simulink model "ZT_VehCtrl_18B_CAN"  (R2018b)
settings: Solver=FixedStepAuto  StartTime=0.0  StopTime=inf  FixedStep=0.005  RelTol=1e-3
InitFcn:
  | mbd_mpc_consistency_checks(bdroot(gcs));
values from neighbouring files (symbols this model uses):
  BatoverTempTh = single(80)    [VCU_INIT.m]
  BRS_PwrValid = single(5)    [VCU_INIT.m]
  BRSEnSpdTh1 = single(10)    [VCU_INIT.m]
  BRSEnSpdTh2 = single(20)    [VCU_INIT.m]
  MCUTempAlarmTh = single (60)    [VCU_INIT.m]
  mps2kmh = single(3.6)    [VCU_INIT.m]
  MtrPwrFac = single(1/9550)    [VCU_INIT.m]
  MtrTempAlarmTh = single (50)    [VCU_INIT.m]
  Padle1Signal1_Th = [PadleSignal1_min,PadleSignal1_max]    [VCU_INIT.m]
  Padle1Signal2_Th = [PadleSignal2_min,PadleSignal2_max]    [VCU_INIT.m]
  PadleSignal1_max = 3.84    [VCU_INIT.m]
  PadleSignal1_min = 0.75    [VCU_INIT.m]
  PadleSignal2_max = 1.92    [VCU_INIT.m]
  PadleSignal2_min = 0.375    [VCU_INIT.m]
  PadleValid = 0.05    [VCU_INIT.m]
  PwrLimFactor = single(0.5)    [VCU_INIT.m]
  Ratio = single(1)    [VCU_INIT.m]
  rpm2mps = single(2*pi/60 * WhlRadius/Ratio)    [VCU_INIT.m]
  SOCLowTh = single(20)    [VCU_INIT.m]
  VehPwrBackwardMax = VehPwrMax * single(0.3)    [VCU_INIT.m]
  VehPwrMax = single(MtrPwrMax * 4)    [VCU_INIT.m]
  VehTrqBackwardMax = VehTrqMax * single(0.3)    [VCU_INIT.m]
  VehTrqMax = single(MtrTrqMax * Ratio *4)    [VCU_INIT.m]
  WhlRadius = single(1)    [VCU_INIT.m]
undefined symbols (not defined in the file or in its folder): Delay_Charge, Delay_Discharge, fifo_0_vect, fifo_1_vect, LQFP, pts1_fifo_0_vect, pts1_fifo_1_vect, pts2_fifo_0_vect, pts2_fifo_1_vect, pts3_fifo_0_vect, pts3_fifo_1_vect, pts4_fifo_0_vect, pts4_fifo_1_vect
libraries: mbd_mpc574x_ec_toolbox x157, canmsglib x74, simulink x38
(part 1 of 12)
settings Model: Creator=DELL  LastModifiedBy=22654
settings SolverCC: AutoInsertRateTranBlk=on
settings DataIOCC: ExternalInput=off  InitialState=off  SaveOutput=off  SignalLogging=off  SaveTime=off  ReturnWorkspaceOutputs=on
settings OptimizationCC: DefaultParameterBehavior=Inlined  DefaultUnderspecifiedDataType=single  EnhancedBackFolding=on  PassReuseOutputArgsAs=Individual arguments  OptimizeBlockOrder=speed  DifferentSizesBufferReuse=on  OptimizationCustomize=off
settings DebuggingCC: InheritedTsInSrcMsg=none  SingleTaskRateTransMsg=error  ParameterTunabilityLossMsg=error  UnconnectedOutputMsg=none  UnconnectedLineMsg=none  UnknownTsInhSupMsg=error  SimStateInterfaceChecksumMismatchMsg=none  UnderSpecifiedDimensionMsg=warning
settings HardwareCC: ProdBitPerPointer=32  ProdBitPerSizeT=32  ProdBitPerPtrDiffT=32  ProdLargestAtomicInteger=Long  ProdLargestAtomicFloat=Double  ProdEndianess=BigEndian  ProdWordSize=32  ProdHWDeviceType=Motorola PowerPC
settings SFSimCC: MATLABDynamicMemAlloc=off
settings RTWCC: SystemTargetFile=mbd_mpc574x.tlc  MakeCommand=mbd_mpc574x_make_rtw  TemplateMakefile=mbd_mpc574x.tmf  Description=Model Based Design Toolbox MPC57xx Code Generation Target  GenerateReport=on  IncludeHyperlinkInReport=on  LaunchReport=on  GenerateTraceInfo=on  GenerateTraceReport=on  GenerateTraceReportSl=on  GenerateTraceReportSf=on  GenerateTraceReportEml=on  RTWCompilerOptimization=on
settings CodeAppCC: ForceParamTrailComments=on  IgnoreCustomStorageClasses=off  MaxIdLength=95  OperatorAnnotations=on  SimulinkDataObjDesc=on  SFDataObjDesc=on  InsertBlockDesc=on
settings STFCustomTargetCC: TargetLangStandard=C99 (ISO)  MultiwordLength=256  CombineOutputUpdateFcns=on  ERTCustomFileBanners=on  SupportNonInlinedSFcns=off  RemoveResetFunc=on  MATLABClassNameForMDSCustomization=Simulink.SoftwareTarget.ERTCustomization  SystemTargetFile=mbd_mpc574x.tlc
settings ERTTargetCC: TargetLangStandard=C99 (ISO)  ParMdlRefBuildCompliant=off  CompOptLevelCompliant=off  ConcurrentExecutionCompliant=off  SupportContinuousTime=on  ModelStepFunctionPrototypeControlCompliant=off  CPPClassGenCompliant=off  UseToolchainInfoCompliant=off  InlinedParameterPlacement=NonHierarchical  ERTSrcFileBannerTemplate=mbd_ert_code_template.cgt  ERTHdrFileBannerTemplate=mbd_ert_code_template.cgt  ERTDataSrcFileTemplate=mbd_ert_code_template.cgt  ERTDataHdrFileTemplate=mbd_ert_code_template.cgt  ERTCustomFileTemplate=example_file_process.tlc

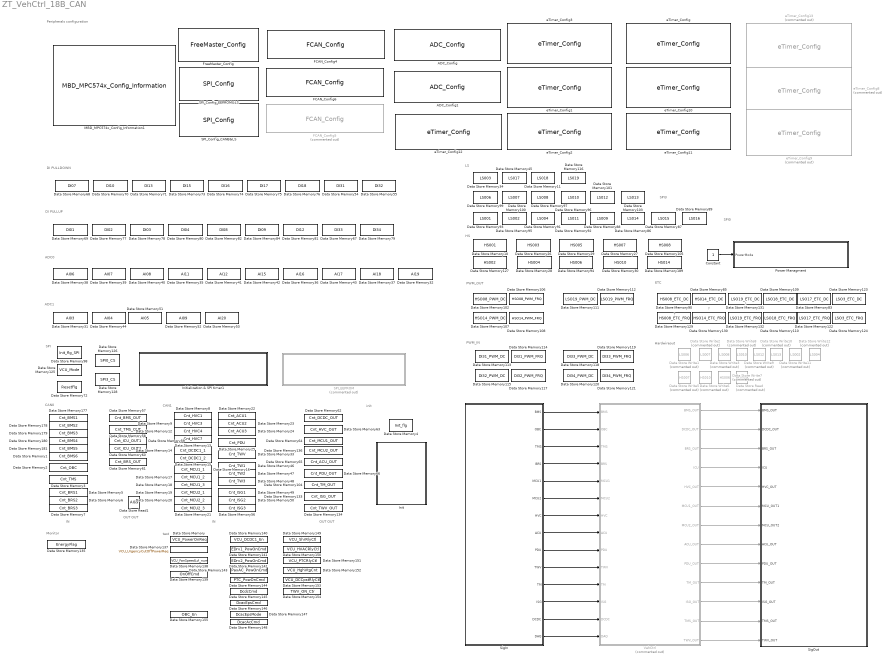
== system ZT_VehCtrl_18B_CAN ==
  note: test
  note: Monitor
  note: IN
  note: CAN1
  note: CAN0
  note: SPI0
  note: SPI3
  note: Hardwireout
  note: ?
  note: LS
  note: ETC
  note: SPI
  note: Peripherals configuration
  note: ADC1
  note: DI PULLUP
  note: PWM_OUT
  note: ADC0
  note: PWM_IN
  note: DI PULLDOWN
  note: ?
  note: ?
  note: HS
  note: init
  note: OUT
      | OUT
  note: IN
  note: OUT
      | OUT
  ADC_Config : mbd_mpc574x_ec_toolbox/Motor Control Blocks/ADC Blocks/ADC_Config  adc_instance=0  adc_mode=One-shot  adc_ctu=Disabled  adc_channels_no_n=10  adc_channel_n_0=PTC2: [ADC0_AN3 | Analog function AN3 of ADC0]  adc_channel_n_1=PTE2: [ADC0_AN5 | Analog function AN5 of ADC0]  adc_channel_n_2=PTB8: [ADC0_AN1 | Analog function AN1 of ADC0]  adc_channel_n_3=PTE7: [ADC0_AN6 | Analog function AN6 of ADC0]  adc_channel_n_4=PTB9: [ADC0_AN11 | Analog function AN11 of ADC0]  adc_channel_n_5=PTC1: [ADC0_AN2 | Analog function AN2 of ADC0]  adc_channel_n_6=PTE4: [ADC0_AN7 | Analog function AN7 of ADC0]  adc_channel_n_7=PTB7: [ADC0_AN0 | Analog function AN0 of ADC0]  adc_channel_n_8=PTE6: [ADC0_AN4 | Analog function AN4 of ADC0]  adc_channel_n_9=PTE5: [ADC0_AN8 | Analog function AN8 of ADC0]  adc_channel_n_10=not available  adc_channel_n_11=not available  adc_channel_n_12=not available  adc_channel_n_13=not available  adc_channel_n_14=not available  adc_channel_n_15=not available  adc_channel_n_16=not available  adc_channel_n_17=not available  adc_channel_n_18=not available  adc_channel_n_19=not available  adc_channel_n_20=not available  adc_channel_n_21=not available  adc_channel_n_22=not available  adc_channel_n_23=not available  adc_channel_n_24=not available  adc_channel_n_25=not available  adc_channel_n_26=not available  adc_channel_n_27=not available  adc_channel_n_28=not available  adc_channel_n_29=not available  adc_channel_n_30=not available  adc_channel_n_31=not available  adc_channel_n_32=not available  adc_channel_n_33=not available  adc_channel_n_34=not available  adc_channel_n_35=not available  adc_channel_n_36=not available  adc_channel_n_37=not available  adc_channel_n_38=not available  adc_channel_n_39=not available  adc_channel_n_40=not available  adc_channel_n_41=not available  adc_channel_n_42=not available  adc_channel_n_43=not available  adc_channel_n_44=not available  adc_channel_n_45=not available  adc_channel_n_46=not available  adc_channel_n_47=not available  show_adv_opts=on  adc_prec=100  adc_presample_0=High voltage ground for ADC  adc_int=100  adc_presample_1=High voltage ground for ADC  adc_ext=100  adc_presample_2=High voltage ground for ADC  adc_clk=Equal to bus clock  adc_ack=off  adc_ext_trigger=External Trigger Disabled  adc_skip_sampling=off  adc_calibration=on  adc_wls=Right  adc_owr=off  adc_inj_trigger=Injected Trigger Disabled  adc_mux_delay=0  adc_decode_delay=0  adc_thr_reg_no=0  adc_upper_value_0=0  adc_lower_value_0=0  adc_upper_value_1=0  adc_lower_value_1=0  adc_upper_value_2=0  adc_lower_value_2=0  adc_upper_value_3=0  adc_lower_value_3=0  adc_upper_value_4=0  adc_lower_value_4=0  adc_upper_value_5=0  adc_lower_value_5=0  adc_upper_value_6=0  adc_lower_value_6=0  adc_upper_value_7=0  adc_lower_value_7=0  adc_upper_value_8=0  adc_lower_value_8=0  adc_upper_value_9=0  adc_lower_value_9=0  adc_upper_value_10=0  adc_lower_value_10=0  adc_upper_value_11=0  adc_lower_value_11=0  adc_upper_value_12=0  adc_lower_value_12=0  adc_upper_value_13=0  adc_lower_value_13=0  adc_upper_value_14=0  adc_lower_value_14=0  adc_upper_value_15=0  adc_lower_value_15=0  adc_wdt_isr_init=off  adc_en_wdt_0=off  adc_th_index_0=0  adc_en_wdt_1=off  adc_th_index_1=0  adc_en_wdt_2=off  adc_th_index_2=0  adc_en_wdt_3=off  adc_th_index_3=0  adc_en_wdt_4=off  adc_th_index_4=0  adc_en_wdt_5=off  adc_th_index_5=0  adc_en_wdt_6=off  adc_th_index_6=0  adc_en_wdt_7=off  adc_th_index_7=0  adc_en_wdt_8=off  adc_th_index_8=0  adc_en_wdt_9=off  adc_th_index_9=0  adc_en_wdt_10=off  adc_th_index_10=0  adc_en_wdt_11=off  adc_th_index_11=0  adc_en_wdt_12=off  adc_th_index_12=0  adc_en_wdt_13=off  adc_th_index_13=0  adc_en_wdt_14=off  adc_th_index_14=0  adc_en_wdt_15=off  adc_th_index_15=0  adc_en_wdt_16=off  adc_th_index_16=0  adc_en_wdt_17=off  adc_th_index_17=0  adc_en_wdt_18=off  adc_th_index_18=0  adc_en_wdt_19=off  adc_th_index_19=0  adc_en_wdt_20=off  adc_th_index_20=0  adc_en_wdt_21=off  adc_th_index_21=0  adc_en_wdt_22=off  adc_th_index_22=0  adc_en_wdt_23=off  adc_th_index_23=0  adc_en_wdt_24=off  adc_th_index_24=0  adc_en_wdt_25=off  adc_th_index_25=0  adc_en_wdt_26=off  adc_th_index_26=0  adc_en_wdt_27=off  adc_th_index_27=0  adc_en_wdt_28=off  adc_th_index_28=0  adc_en_wdt_29=off  adc_th_index_29=0  adc_en_wdt_30=off  adc_th_index_30=0  adc_en_wdt_31=off  adc_th_index_31=0  adc_en_wdt_32=off  adc_th_index_32=0  adc_en_wdt_33=off  adc_th_index_33=0  adc_en_wdt_34=off  adc_th_index_34=0  adc_en_wdt_35=off  adc_th_index_35=0  adc_en_wdt_36=off  adc_th_index_36=0  adc_en_wdt_37=off  adc_th_index_37=0  adc_en_wdt_38=off  adc_th_index_38=0  adc_en_wdt_39=off  adc_th_index_39=0  adc_en_wdt_40=off  adc_th_index_40=0  adc_en_wdt_41=off  adc_th_index_41=0  adc_en_wdt_42=off  adc_th_index_42=0  adc_en_wdt_43=off  adc_th_index_43=0  adc_en_wdt_44=off  adc_th_index_44=0  adc_en_wdt_45=off  adc_th_index_45=0  adc_en_wdt_46=off  adc_th_index_46=0  adc_en_wdt_47=off  adc_th_index_47=0
  ADC_Config1 : mbd_mpc574x_ec_toolbox/Motor Control Blocks/ADC Blocks/ADC_Config  adc_instance=1  adc_mode=One-shot  adc_ctu=Disabled  adc_channels_no_n=5  adc_channel_n_0=PTC0: [ADC1_AN3 | Analog function AN3 of ADC1]  adc_channel_n_1=PTE11: [ADC1_AN4 | Analog function AN4 of ADC1]  adc_channel_n_2=PTB15: [ADC1_AN2 | Analog function AN2 of ADC1]  adc_channel_n_3=PTE0: [ADC1_AN5 | Analog function AN5 of ADC1]  adc_channel_n_4=PTB14: [ADC1_AN1 | Analog function AN1 of ADC1]  adc_channel_n_5=not available  adc_channel_n_6=not available  adc_channel_n_7=not available  adc_channel_n_8=not available  adc_channel_n_9=not available  adc_channel_n_10=not available  adc_channel_n_11=not available  adc_channel_n_12=not available  adc_channel_n_13=not available  adc_channel_n_14=not available  adc_channel_n_15=not available  adc_channel_n_16=not available  adc_channel_n_17=not available  adc_channel_n_18=not available  adc_channel_n_19=not available  adc_channel_n_20=not available  adc_channel_n_21=not available  adc_channel_n_22=not available  adc_channel_n_23=not available  adc_channel_n_24=not available  adc_channel_n_25=not available  adc_channel_n_26=not available  adc_channel_n_27=not available  adc_channel_n_28=not available  adc_channel_n_29=not available  adc_channel_n_30=not available  adc_channel_n_31=not available  adc_channel_n_32=not available  adc_channel_n_33=not available  adc_channel_n_34=not available  adc_channel_n_35=not available  adc_channel_n_36=not available  adc_channel_n_37=not available  adc_channel_n_38=not available  adc_channel_n_39=not available  adc_channel_n_40=not available  adc_channel_n_41=not available  adc_channel_n_42=not available  adc_channel_n_43=not available  adc_channel_n_44=not available  adc_channel_n_45=not available  adc_channel_n_46=not available  adc_channel_n_47=not available  show_adv_opts=on  adc_prec=100  adc_presample_0=High voltage ground for ADC  adc_int=100  adc_presample_1=High voltage ground for ADC  adc_ext=100  adc_presample_2=High voltage ground for ADC  adc_clk=Equal to bus clock  adc_ack=off  adc_ext_trigger=External Trigger Disabled  adc_skip_sampling=off  adc_calibration=on  adc_wls=Right  adc_owr=off  adc_inj_trigger=Injected Trigger Disabled  adc_mux_delay=0  adc_decode_delay=0  adc_thr_reg_no=0  adc_upper_value_0=0  adc_lower_value_0=0  adc_upper_value_1=0  adc_lower_value_1=0  adc_upper_value_2=0  adc_lower_value_2=0  adc_upper_value_3=0  adc_lower_value_3=0  adc_upper_value_4=0  adc_lower_value_4=0  adc_upper_value_5=0  adc_lower_value_5=0  adc_upper_value_6=0  adc_lower_value_6=0  adc_upper_value_7=0  adc_lower_value_7=0  adc_upper_value_8=0  adc_lower_value_8=0  adc_upper_value_9=0  adc_lower_value_9=0  adc_upper_value_10=0  adc_lower_value_10=0  adc_upper_value_11=0  adc_lower_value_11=0  adc_upper_value_12=0  adc_lower_value_12=0  adc_upper_value_13=0  adc_lower_value_13=0  adc_upper_value_14=0  adc_lower_value_14=0  adc_upper_value_15=0  adc_lower_value_15=0  adc_wdt_isr_init=off  adc_en_wdt_0=off  adc_th_index_0=0  adc_en_wdt_1=off  adc_th_index_1=0  adc_en_wdt_2=off  adc_th_index_2=0  adc_en_wdt_3=off  adc_th_index_3=0  adc_en_wdt_4=off  adc_th_index_4=0  adc_en_wdt_5=off  adc_th_index_5=0  adc_en_wdt_6=off  adc_th_index_6=0  adc_en_wdt_7=off  adc_th_index_7=0  adc_en_wdt_8=off  adc_th_index_8=0  adc_en_wdt_9=off  adc_th_index_9=0  adc_en_wdt_10=off  adc_th_index_10=0  adc_en_wdt_11=off  adc_th_index_11=0  adc_en_wdt_12=off  adc_th_index_12=0  adc_en_wdt_13=off  adc_th_index_13=0  adc_en_wdt_14=off  adc_th_index_14=0  adc_en_wdt_15=off  adc_th_index_15=0  adc_en_wdt_16=off  adc_th_index_16=0  adc_en_wdt_17=off  adc_th_index_17=0  adc_en_wdt_18=off  adc_th_index_18=0  adc_en_wdt_19=off  adc_th_index_19=0  adc_en_wdt_20=off  adc_th_index_20=0  adc_en_wdt_21=off  adc_th_index_21=0  adc_en_wdt_22=off  adc_th_index_22=0  adc_en_wdt_23=off  adc_th_index_23=0  adc_en_wdt_24=off  adc_th_index_24=0  adc_en_wdt_25=off  adc_th_index_25=0  adc_en_wdt_26=off  adc_th_index_26=0  adc_en_wdt_27=off  adc_th_index_27=0  adc_en_wdt_28=off  adc_th_index_28=0  adc_en_wdt_29=off  adc_th_index_29=0  adc_en_wdt_30=off  adc_th_index_30=0  adc_en_wdt_31=off  adc_th_index_31=0  adc_en_wdt_32=off  adc_th_index_32=0  adc_en_wdt_33=off  adc_th_index_33=0  adc_en_wdt_34=off  adc_th_index_34=0  adc_en_wdt_35=off  adc_th_index_35=0  adc_en_wdt_36=off  adc_th_index_36=0  adc_en_wdt_37=off  adc_th_index_37=0  adc_en_wdt_38=off  adc_th_index_38=0  adc_en_wdt_39=off  adc_th_index_39=0  adc_en_wdt_40=off  adc_th_index_40=0  adc_en_wdt_41=off  adc_th_index_41=0  adc_en_wdt_42=off  adc_th_index_42=0  adc_en_wdt_43=off  adc_th_index_43=0  adc_en_wdt_44=off  adc_th_index_44=0  adc_en_wdt_45=off  adc_th_index_45=0  adc_en_wdt_46=off  adc_th_index_46=0  adc_en_wdt_47=off  adc_th_index_47=0
  Constant : Constant
  Data Store Memory : DataStoreMemory  DataStoreName=VCU_PowerOnReq  ReadBeforeWriteMsg=warning  WriteAfterWriteMsg=warning  WriteAfterReadMsg=warning  ShowAdditionalParam=off  OutDataTypeStr=boolean
      settings: RTWStateStorageClass=ExportedGlobal
  Data Store Memory1 : DataStoreMemory  DataStoreName=Cnt_BMS6  ReadBeforeWriteMsg=warning  WriteAfterWriteMsg=warning  WriteAfterReadMsg=warning  ShowAdditionalParam=off  OutDataTypeStr=uint8
      settings: RTWStateStorageClass=ExportedGlobal
  Data Store Memory10 : DataStoreMemory  DataStoreName=HS001  ReadBeforeWriteMsg=warning  WriteAfterWriteMsg=warning  WriteAfterReadMsg=warning  ShowAdditionalParam=off  OutDataTypeStr=boolean
  Data Store Memory100 : DataStoreMemory  DataStoreName=LS007  ReadBeforeWriteMsg=warning  WriteAfterWriteMsg=warning  WriteAfterReadMsg=warning  ShowAdditionalParam=off  OutDataTypeStr=boolean
      settings: RTWStateStorageClass=ExportedGlobal
  Data Store Memory101 : DataStoreMemory  DataStoreName=LS012  ReadBeforeWriteMsg=warning  WriteAfterWriteMsg=warning  WriteAfterReadMsg=warning  ShowAdditionalParam=off  OutDataTypeStr=boolean
      settings: RTWStateStorageClass=ExportedGlobal
  Data Store Memory102 : DataStoreMemory  DataStoreName=HSO08_PWM_DC  ReadBeforeWriteMsg=warning  WriteAfterWriteMsg=warning  WriteAfterReadMsg=warning  ShowAdditionalParam=off  OutMin=0  OutMax=1  OutDataTypeStr=single
  Data Store Memory103 : DataStoreMemory  DataStoreName=LS013  ReadBeforeWriteMsg=warning  WriteAfterWriteMsg=warning  WriteAfterReadMsg=warning  ShowAdditionalParam=off  OutDataTypeStr=boolean
      settings: RTWStateStorageClass=ExportedGlobal
  Data Store Memory104 : DataStoreMemory  DataStoreName=Cnt_TM_OUT  ReadBeforeWriteMsg=warning  WriteAfterWriteMsg=warning  WriteAfterReadMsg=warning  ShowAdditionalParam=off  OutDataTypeStr=uint8
      settings: RTWStateStorageClass=ExportedGlobal
  Data Store Memory105 : DataStoreMemory  DataStoreName=HS008  ReadBeforeWriteMsg=warning  WriteAfterWriteMsg=warning  WriteAfterReadMsg=warning  ShowAdditionalParam=off  OutDataTypeStr=boolean
  Data Store Memory106 : DataStoreMemory  DataStoreName=HSO08_PWM_FRQ  ReadBeforeWriteMsg=warning  WriteAfterWriteMsg=warning  WriteAfterReadMsg=warning  InitialValue=200  ShowAdditionalParam=off  OutMin=20  OutMax=20000  OutDataTypeStr=single
  Data Store Memory107 : DataStoreMemory  DataStoreName=HSO14_PWM_DC  ReadBeforeWriteMsg=warning  WriteAfterWriteMsg=warning  WriteAfterReadMsg=warning  ShowAdditionalParam=off  OutMin=0  OutMax=1  OutDataTypeStr=single
  Data Store Memory108 : DataStoreMemory  DataStoreName=HSO14_PWM_FRQ  ReadBeforeWriteMsg=warning  WriteAfterWriteMsg=warning  WriteAfterReadMsg=warning  InitialValue=200  ShowAdditionalParam=off  OutMin=20  OutMax=20000  OutDataTypeStr=single
  Data Store Memory109 : DataStoreMemory  DataStoreName=LSO18_ETC_DC  ReadBeforeWriteMsg=warning  WriteAfterWriteMsg=warning  WriteAfterReadMsg=warning  ShowAdditionalParam=off  OutMin=0  OutMax=1  OutDataTypeStr=single
  Data Store Memory11 : DataStoreMemory  DataStoreName=LS018  ReadBeforeWriteMsg=warning  WriteAfterWriteMsg=warning  WriteAfterReadMsg=warning  ShowAdditionalParam=off  OutDataTypeStr=boolean
      settings: RTWStateStorageClass=ExportedGlobal
  Data Store Memory110 : DataStoreMemory  DataStoreName=LSO18_ETC_FRQ  ReadBeforeWriteMsg=warning  WriteAfterWriteMsg=warning  WriteAfterReadMsg=warning  InitialValue=200  ShowAdditionalParam=off  OutMin=20  OutMax=20000  OutDataTypeStr=single
  Data Store Memory111 : DataStoreMemory  DataStoreName=LSO19_PWM_DC  ReadBeforeWriteMsg=warning  WriteAfterWriteMsg=warning  WriteAfterReadMsg=warning  ShowAdditionalParam=off  OutMin=0  OutMax=1  OutDataTypeStr=single
  Data Store Memory112 : DataStoreMemory  DataStoreName=LSO19_PWM_FRQ  ReadBeforeWriteMsg=warning  WriteAfterWriteMsg=warning  WriteAfterReadMsg=warning  InitialValue=200  ShowAdditionalParam=off  OutMin=20  OutMax=20000  OutDataTypeStr=single
  Data Store Memory113 : DataStoreMemory  DataStoreName=DI31_PWM_DC  ReadBeforeWriteMsg=warning  WriteAfterWriteMsg=warning  WriteAfterReadMsg=warning  InitialValue=0.5  ShowAdditionalParam=off  OutDataTypeStr=single
  Data Store Memory114 : DataStoreMemory  DataStoreName=DI31_PWM_FRQ  ReadBeforeWriteMsg=warning  WriteAfterWriteMsg=warning  WriteAfterReadMsg=warning  InitialValue=200  ShowAdditionalParam=off  OutDataTypeStr=single
  Data Store Memory115 : DataStoreMemory  DataStoreName=DI32_PWM_DC  ReadBeforeWriteMsg=warning  WriteAfterWriteMsg=warning  WriteAfterReadMsg=warning  InitialValue=0.5  ShowAdditionalParam=off  OutDataTypeStr=single
  Data Store Memory116 : DataStoreMemory  DataStoreName=LS019  ReadBeforeWriteMsg=warning  WriteAfterWriteMsg=warning  WriteAfterReadMsg=warning  ShowAdditionalParam=off  OutDataTypeStr=boolean
      settings: RTWStateStorageClass=ExportedGlobal
  Data Store Memory117 : DataStoreMemory  DataStoreName=DI32_PWM_FRQ  ReadBeforeWriteMsg=warning  WriteAfterWriteMsg=warning  WriteAfterReadMsg=warning  InitialValue=200  ShowAdditionalParam=off  OutDataTypeStr=single
  Data Store Memory118 : DataStoreMemory  DataStoreName=DI33_PWM_DC  ReadBeforeWriteMsg=warning  WriteAfterWriteMsg=warning  WriteAfterReadMsg=warning  InitialValue=0.5  ShowAdditionalParam=off  OutDataTypeStr=single
  Data Store Memory119 : DataStoreMemory  DataStoreName=DI33_PWM_FRQ  ReadBeforeWriteMsg=warning  WriteAfterWriteMsg=warning  WriteAfterReadMsg=warning  InitialValue=200  ShowAdditionalParam=off  OutDataTypeStr=single
  Data Store Memory12 : DataStoreMemory  DataStoreName=Cnt_HVC4  ReadBeforeWriteMsg=warning  WriteAfterWriteMsg=warning  WriteAfterReadMsg=warning  ShowAdditionalParam=off  OutDataTypeStr=uint8
      settings: RTWStateStorageClass=ExportedGlobal
  Data Store Memory120 : DataStoreMemory  DataStoreName=DI34_PWM_DC  ReadBeforeWriteMsg=warning  WriteAfterWriteMsg=warning  WriteAfterReadMsg=warning  InitialValue=0.5  ShowAdditionalParam=off  OutDataTypeStr=single
  Data Store Memory121 : DataStoreMemory  DataStoreName=DI34_PWM_FRQ  ReadBeforeWriteMsg=warning  WriteAfterWriteMsg=warning  WriteAfterReadMsg=warning  InitialValue=200  ShowAdditionalParam=off  OutDataTypeStr=single
  Data Store Memory122 : DataStoreMemory  DataStoreName=LSO17_ETC_FRQ  ReadBeforeWriteMsg=warning  WriteAfterWriteMsg=warning  WriteAfterReadMsg=warning  InitialValue=200  ShowAdditionalParam=off  OutMin=20  OutMax=20000  OutDataTypeStr=single
  Data Store Memory123 : DataStoreMemory  DataStoreName=LSO3_ETC_DC  ReadBeforeWriteMsg=warning  WriteAfterWriteMsg=warning  WriteAfterReadMsg=warning  ShowAdditionalParam=off  OutMin=0  OutMax=1  OutDataTypeStr=single
  Data Store Memory124 : DataStoreMemory  DataStoreName=LSO3_ETC_FRQ  ReadBeforeWriteMsg=warning  WriteAfterWriteMsg=warning  WriteAfterReadMsg=warning  InitialValue=200  ShowAdditionalParam=off  OutMin=20  OutMax=20000  OutDataTypeStr=single
  Data Store Memory125 : DataStoreMemory  DataStoreName=VCU_Mode  ReadBeforeWriteMsg=warning  WriteAfterWriteMsg=warning  WriteAfterReadMsg=warning  ShowAdditionalParam=off  OutDataTypeStr=uint8
      settings: RTWStateStorageClass=ExportedGlobal
  Data Store Memory126 : DataStoreMemory  DataStoreName=SPI0_CS  ReadBeforeWriteMsg=warning  WriteAfterWriteMsg=warning  WriteAfterReadMsg=warning  ShowAdditionalParam=off  OutDataTypeStr=boolean
  Data Store Memory127 : DataStoreMemory  DataStoreName=HS002  ReadBeforeWriteMsg=warning  WriteAfterWriteMsg=warning  WriteAfterReadMsg=warning  ShowAdditionalParam=off  OutDataTypeStr=boolean
  Data Store Memory128 : DataStoreMemory  DataStoreName=SPI3_CS  ReadBeforeWriteMsg=warning  WriteAfterWriteMsg=warning  WriteAfterReadMsg=warning  ShowAdditionalParam=off  OutDataTypeStr=boolean
  Data Store Memory129 : DataStoreMemory  DataStoreName=HS008_ETC_FRQ  ReadBeforeWriteMsg=warning  WriteAfterWriteMsg=warning  WriteAfterReadMsg=warning  InitialValue=200  ShowAdditionalParam=off  OutMin=20  OutMax=20000  OutDataTypeStr=single
  Data Store Memory13 : DataStoreMemory  DataStoreName=Cnt_HVC7  ReadBeforeWriteMsg=warning  WriteAfterWriteMsg=warning  WriteAfterReadMsg=warning  ShowAdditionalParam=off  OutDataTypeStr=uint8
      settings: RTWStateStorageClass=ExportedGlobal
  Data Store Memory130 : DataStoreMemory  DataStoreName=HSO14_ETC_FRQ  ReadBeforeWriteMsg=warning  WriteAfterWriteMsg=warning  WriteAfterReadMsg=warning  InitialValue=200  ShowAdditionalParam=off  OutMin=20  OutMax=20000  OutDataTypeStr=single
  Data Store Memory131 : DataStoreMemory  DataStoreName=LSO19_ETC_DC  ReadBeforeWriteMsg=warning  WriteAfterWriteMsg=warning  WriteAfterReadMsg=warning  ShowAdditionalParam=off  OutMin=0  OutMax=1  OutDataTypeStr=single
  Data Store Memory132 : DataStoreMemory  DataStoreName=LSO19_ETC_FRQ  ReadBeforeWriteMsg=warning  WriteAfterWriteMsg=warning  WriteAfterReadMsg=warning  InitialValue=200  ShowAdditionalParam=off  OutMin=20  OutMax=20000  OutDataTypeStr=single
  Data Store Memory133 : DataStoreMemory  DataStoreName=Cnt_ISG_OUT  ReadBeforeWriteMsg=warning  WriteAfterWriteMsg=warning  WriteAfterReadMsg=warning  ShowAdditionalParam=off  OutDataTypeStr=uint8
      settings: RTWStateStorageClass=ExportedGlobal
  Data Store Memory134 : DataStoreMemory  DataStoreName=Cnt_TWV_OUT  ReadBeforeWriteMsg=warning  WriteAfterWriteMsg=warning  WriteAfterReadMsg=warning  ShowAdditionalParam=off  OutDataTypeStr=uint8
      settings: RTWStateStorageClass=ExportedGlobal
  Data Store Memory135 : DataStoreMemory  DataStoreName=EnergyFlag  ReadBeforeWriteMsg=warning  WriteAfterWriteMsg=warning  WriteAfterReadMsg=warning  ShowAdditionalParam=off  OutDataTypeStr=uint8
      settings: RTWStateStorageClass=ExportedGlobal
  Data Store Memory136 : DataStoreMemory  DataStoreName=Cnt_MCU2_OUT  ReadBeforeWriteMsg=warning  WriteAfterWriteMsg=warning  WriteAfterReadMsg=warning  ShowAdditionalParam=off  OutDataTypeStr=uint8
      settings: RTWStateStorageClass=ExportedGlobal
  Data Store Memory137 : DataStoreMemory  DataStoreName=VCU_UrgencyCutOffPowerReq  ReadBeforeWriteMsg=warning  WriteAfterWriteMsg=warning  WriteAfterReadMsg=warning  ShowAdditionalParam=off  OutDataTypeStr=boolean
      settings: RTWStateStorageClass=ExportedGlobal
  Data Store Memory138 : DataStoreMemory  DataStoreName=VCU_FanSpeedLvl_num  ReadBeforeWriteMsg=warning  WriteAfterWriteMsg=warning  WriteAfterReadMsg=warning  ShowAdditionalParam=off  OutDataTypeStr=single
      settings: RTWStateStorageClass=ExportedGlobal
  Data Store Memory139 : DataStoreMemory  DataStoreName=OnOffCmd  ReadBeforeWriteMsg=warning  WriteAfterWriteMsg=warning  WriteAfterReadMsg=warning  ShowAdditionalParam=off  OutDataTypeStr=boolean
      settings: RTWStateStorageClass=ExportedGlobal
  Data Store Memory14 : DataStoreMemory  DataStoreName=Cnt_DCDC1_1  ReadBeforeWriteMsg=warning  WriteAfterWriteMsg=warning  WriteAfterReadMsg=warning  ShowAdditionalParam=off  OutDataTypeStr=uint8
      settings: RTWStateStorageClass=ExportedGlobal
  Data Store Memory140 : DataStoreMemory  DataStoreName=VCU_DCDC1_En  ReadBeforeWriteMsg=warning  WriteAfterWriteMsg=warning  WriteAfterReadMsg=warning  ShowAdditionalParam=off  OutDataTypeStr=single
      settings: RTWStateStorageClass=ExportedGlobal
  Data Store Memory141 : DataStoreMemory  DataStoreName=EDrv1_PowOnCmd  ReadBeforeWriteMsg=warning  WriteAfterWriteMsg=warning  WriteAfterReadMsg=warning  ShowAdditionalParam=off  OutDataTypeStr=boolean
      settings: RTWStateStorageClass=ExportedGlobal
  Data Store Memory142 : DataStoreMemory  DataStoreName=EDrv2_PowOnCmd  ReadBeforeWriteMsg=warning  WriteAfterWriteMsg=warning  WriteAfterReadMsg=warning  ShowAdditionalParam=off  OutDataTypeStr=boolean
      settings: RTWStateStorageClass=ExportedGlobal
  Data Store Memory143 : DataStoreMemory  DataStoreName=PaxAC_PowOnCmd  ReadBeforeWriteMsg=warning  WriteAfterWriteMsg=warning  WriteAfterReadMsg=warning  ShowAdditionalParam=off  OutDataTypeStr=boolean
      settings: RTWStateStorageClass=ExportedGlobal
  Data Store Memory144 : DataStoreMemory  DataStoreName=PTC_PowOnCmd  ReadBeforeWriteMsg=warning  WriteAfterWriteMsg=warning  WriteAfterReadMsg=warning  ShowAdditionalParam=off  OutDataTypeStr=boolean
      settings: RTWStateStorageClass=ExportedGlobal
  Data Store Memory145 : DataStoreMemory  DataStoreName=DcdcCmd  ReadBeforeWriteMsg=warning  WriteAfterWriteMsg=warning  WriteAfterReadMsg=warning  ShowAdditionalParam=off  OutDataTypeStr=single
      settings: RTWStateStorageClass=ExportedGlobal
  Data Store Memory146 : DataStoreMemory  DataStoreName=DcacEpsCmd  ReadBeforeWriteMsg=warning  WriteAfterWriteMsg=warning  WriteAfterReadMsg=warning  ShowAdditionalParam=off  OutDataTypeStr=single
      settings: RTWStateStorageClass=ExportedGlobal
  Data Store Memory147 : DataStoreMemory  DataStoreName=DcacEpsMode  ReadBeforeWriteMsg=warning  WriteAfterWriteMsg=warning  WriteAfterReadMsg=warning  ShowAdditionalParam=off  OutDataTypeStr=single
      settings: RTWStateStorageClass=ExportedGlobal
  Data Store Memory148 : DataStoreMemory  DataStoreName=DcacAcCmd  ReadBeforeWriteMsg=warning  WriteAfterWriteMsg=warning  WriteAfterReadMsg=warning  ShowAdditionalParam=off  OutDataTypeStr=single
      settings: RTWStateStorageClass=ExportedGlobal
  Data Store Memory149 : DataStoreMemory  DataStoreName=VCU_ShrRlyCtl  ReadBeforeWriteMsg=warning  WriteAfterWriteMsg=warning  WriteAfterReadMsg=warning  ShowAdditionalParam=off  OutDataTypeStr=single
      settings: RTWStateStorageClass=ExportedGlobal
  Data Store Memory15 : DataStoreMemory  DataStoreName=Cnt_DCDC1_2  ReadBeforeWriteMsg=warning  WriteAfterWriteMsg=warning  WriteAfterReadMsg=warning  ShowAdditionalParam=off  OutDataTypeStr=uint8
      settings: RTWStateStorageClass=ExportedGlobal
  Data Store Memory150 : DataStoreMemory  DataStoreName=VCU_HVACRlyCtl  ReadBeforeWriteMsg=warning  WriteAfterWriteMsg=warning  WriteAfterReadMsg=warning  ShowAdditionalParam=off  OutDataTypeStr=single
      settings: RTWStateStorageClass=ExportedGlobal
  Data Store Memory151 : DataStoreMemory  DataStoreName=VCU_PTCRlyCtl  ReadBeforeWriteMsg=warning  WriteAfterWriteMsg=warning  WriteAfterReadMsg=warning  ShowAdditionalParam=off  OutDataTypeStr=single
      settings: RTWStateStorageClass=ExportedGlobal
  Data Store Memory152 : DataStoreMemory  DataStoreName=VCU_HghVtgCnt  ReadBeforeWriteMsg=warning  WriteAfterWriteMsg=warning  WriteAfterReadMsg=warning  ShowAdditionalParam=off  OutDataTypeStr=single
      settings: RTWStateStorageClass=ExportedGlobal
  Data Store Memory153 : DataStoreMemory  DataStoreName=VCU_DCCpstRlyCtl  ReadBeforeWriteMsg=warning  WriteAfterWriteMsg=warning  WriteAfterReadMsg=warning  ShowAdditionalParam=off  OutDataTypeStr=single
      settings: RTWStateStorageClass=ExportedGlobal
  Data Store Memory154 : DataStoreMemory  DataStoreName=TWV_ON_Ctr  ReadBeforeWriteMsg=warning  WriteAfterWriteMsg=warning  WriteAfterReadMsg=warning  ShowAdditionalParam=off  OutDataTypeStr=single
      settings: RTWStateStorageClass=ExportedGlobal
  Data Store Memory155 : DataStoreMemory  DataStoreName=OBC_En  ReadBeforeWriteMsg=warning  WriteAfterWriteMsg=warning  WriteAfterReadMsg=warning  ShowAdditionalParam=off  OutDataTypeStr=boolean
      settings: RTWStateStorageClass=ExportedGlobal
  Data Store Memory16 : DataStoreMemory  DataStoreName=Cnt_MCU1_1  ReadBeforeWriteMsg=warning  WriteAfterWriteMsg=warning  WriteAfterReadMsg=warning  ShowAdditionalParam=off  OutDataTypeStr=uint8
      settings: RTWStateStorageClass=ExportedGlobal
  Data Store Memory17 : DataStoreMemory  DataStoreName=Cnt_MCU1_2  ReadBeforeWriteMsg=warning  WriteAfterWriteMsg=warning  WriteAfterReadMsg=warning  ShowAdditionalParam=off  OutDataTypeStr=uint8
      settings: RTWStateStorageClass=ExportedGlobal
  Data Store Memory177 : DataStoreMemory  DataStoreName=Cnt_BMS1  ReadBeforeWriteMsg=warning  WriteAfterWriteMsg=warning  WriteAfterReadMsg=warning  ShowAdditionalParam=off  OutDataTypeStr=uint8
      settings: RTWStateStorageClass=ExportedGlobal
  Data Store Memory178 : DataStoreMemory  DataStoreName=Cnt_BMS2  ReadBeforeWriteMsg=warning  WriteAfterWriteMsg=warning  WriteAfterReadMsg=warning  ShowAdditionalParam=off  OutDataTypeStr=uint8
      settings: RTWStateStorageClass=ExportedGlobal
  Data Store Memory179 : DataStoreMemory  DataStoreName=Cnt_BMS3  ReadBeforeWriteMsg=warning  WriteAfterWriteMsg=warning  WriteAfterReadMsg=warning  ShowAdditionalParam=off  OutDataTypeStr=uint8
      settings: RTWStateStorageClass=ExportedGlobal
  Data Store Memory18 : DataStoreMemory  DataStoreName=Cnt_MCU1_3  ReadBeforeWriteMsg=warning  WriteAfterWriteMsg=warning  WriteAfterReadMsg=warning  ShowAdditionalParam=off  OutDataTypeStr=uint8
      settings: RTWStateStorageClass=ExportedGlobal
  Data Store Memory180 : DataStoreMemory  DataStoreName=Cnt_BMS4  ReadBeforeWriteMsg=warning  WriteAfterWriteMsg=warning  WriteAfterReadMsg=warning  ShowAdditionalParam=off  OutDataTypeStr=uint8
      settings: RTWStateStorageClass=ExportedGlobal
  Data Store Memory181 : DataStoreMemory  DataStoreName=Cnt_BMS5  ReadBeforeWriteMsg=warning  WriteAfterWriteMsg=warning  WriteAfterReadMsg=warning  ShowAdditionalParam=off  OutDataTypeStr=uint8
      settings: RTWStateStorageClass=ExportedGlobal
  Data Store Memory189 : DataStoreMemory  DataStoreName=HS014  ReadBeforeWriteMsg=warning  WriteAfterWriteMsg=warning  WriteAfterReadMsg=warning  ShowAdditionalParam=off  OutDataTypeStr=boolean
  Data Store Memory19 : DataStoreMemory  DataStoreName=Cnt_MCU2_1  ReadBeforeWriteMsg=warning  WriteAfterWriteMsg=warning  WriteAfterReadMsg=warning  ShowAdditionalParam=off  OutDataTypeStr=uint8
      settings: RTWStateStorageClass=ExportedGlobal
  Data Store Memory2 : DataStoreMemory  DataStoreName=Cnt_OBC  ReadBeforeWriteMsg=warning  WriteAfterWriteMsg=warning  WriteAfterReadMsg=warning  ShowAdditionalParam=off  OutDataTypeStr=uint8
      settings: RTWStateStorageClass=ExportedGlobal
  Data Store Memory20 : DataStoreMemory  DataStoreName=Cnt_MCU2_2  ReadBeforeWriteMsg=warning  WriteAfterWriteMsg=warning  WriteAfterReadMsg=warning  ShowAdditionalParam=off  OutDataTypeStr=uint8
      settings: RTWStateStorageClass=ExportedGlobal
  Data Store Memory21 : DataStoreMemory  DataStoreName=Cnt_MCU2_3  ReadBeforeWriteMsg=warning  WriteAfterWriteMsg=warning  WriteAfterReadMsg=warning  ShowAdditionalParam=off  OutDataTypeStr=uint8
      settings: RTWStateStorageClass=ExportedGlobal
  Data Store Memory22 : DataStoreMemory  DataStoreName=Cnt_ACU1  ReadBeforeWriteMsg=warning  WriteAfterWriteMsg=warning  WriteAfterReadMsg=warning  ShowAdditionalParam=off  OutDataTypeStr=uint8
      settings: RTWStateStorageClass=ExportedGlobal
  Data Store Memory23 : DataStoreMemory  DataStoreName=Cnt_ACU2  ReadBeforeWriteMsg=warning  WriteAfterWriteMsg=warning  WriteAfterReadMsg=warning  ShowAdditionalParam=off  OutDataTypeStr=uint8
      settings: RTWStateStorageClass=ExportedGlobal
  Data Store Memory24 : DataStoreMemory  DataStoreName=Cnt_ACU3  ReadBeforeWriteMsg=warning  WriteAfterWriteMsg=warning  WriteAfterReadMsg=warning  ShowAdditionalParam=off  OutDataTypeStr=uint8
      settings: RTWStateStorageClass=ExportedGlobal
  Data Store Memory25 : DataStoreMemory  DataStoreName=Cnt_PDU  ReadBeforeWriteMsg=warning  WriteAfterWriteMsg=warning  WriteAfterReadMsg=warning  ShowAdditionalParam=off  OutDataTypeStr=uint8
      settings: RTWStateStorageClass=ExportedGlobal
  Data Store Memory26 : DataStoreMemory  DataStoreName=HS003  ReadBeforeWriteMsg=warning  WriteAfterWriteMsg=warning  WriteAfterReadMsg=warning  ShowAdditionalParam=off  OutDataTypeStr=boolean
  Data Store Memory27 : DataStoreMemory  DataStoreName=HS007  ReadBeforeWriteMsg=warning  WriteAfterWriteMsg=warning  WriteAfterReadMsg=warning  ShowAdditionalParam=off  OutDataTypeStr=boolean
  Data Store Memory28 : DataStoreMemory  DataStoreName=HS004  ReadBeforeWriteMsg=warning  WriteAfterWriteMsg=warning  WriteAfterReadMsg=warning  ShowAdditionalParam=off  OutDataTypeStr=boolean
  Data Store Memory29 : DataStoreMemory  DataStoreName=HS005  ReadBeforeWriteMsg=warning  WriteAfterWriteMsg=warning  WriteAfterReadMsg=warning  ShowAdditionalParam=off  OutDataTypeStr=boolean
  Data Store Memory3 : DataStoreMemory  DataStoreName=Cnt_TMS  ReadBeforeWriteMsg=warning  WriteAfterWriteMsg=warning  WriteAfterReadMsg=warning  ShowAdditionalParam=off  OutDataTypeStr=uint8
      settings: RTWStateStorageClass=ExportedGlobal
  Data Store Memory30 : DataStoreMemory  DataStoreName=HS010  ReadBeforeWriteMsg=warning  WriteAfterWriteMsg=warning  WriteAfterReadMsg=warning  ShowAdditionalParam=off  OutDataTypeStr=boolean
  Data Store Memory31 : DataStoreMemory  DataStoreName=AI03  ReadBeforeWriteMsg=warning  WriteAfterWriteMsg=warning  WriteAfterReadMsg=warning  ShowAdditionalParam=off  OutDataTypeStr=single
  Data Store Memory32 : DataStoreMemory  DataStoreName=AI19  ReadBeforeWriteMsg=warning  WriteAfterWriteMsg=warning  WriteAfterReadMsg=warning  ShowAdditionalParam=off  OutDataTypeStr=single
  Data Store Memory33 : DataStoreMemory  DataStoreName=Cnt_TWV  ReadBeforeWriteMsg=warning  WriteAfterWriteMsg=warning  WriteAfterReadMsg=warning  ShowAdditionalParam=off  OutDataTypeStr=uint8
      settings: RTWStateStorageClass=ExportedGlobal
  Data Store Memory34 : DataStoreMemory  DataStoreName=LS003  ReadBeforeWriteMsg=warning  WriteAfterWriteMsg=warning  WriteAfterReadMsg=warning  ShowAdditionalParam=off  OutDataTypeStr=boolean
      settings: RTWStateStorageClass=ExportedGlobal
  Data Store Memory35 : DataStoreMemory  DataStoreName=AI11  ReadBeforeWriteMsg=warning  WriteAfterWriteMsg=warning  WriteAfterReadMsg=warning  ShowAdditionalParam=off  OutDataTypeStr=single
  Data Store Memory36 : DataStoreMemory  DataStoreName=AI16  ReadBeforeWriteMsg=warning  WriteAfterWriteMsg=warning  WriteAfterReadMsg=warning  ShowAdditionalParam=off  OutDataTypeStr=single
  Data Store Memory37 : DataStoreMemory  DataStoreName=AI18  ReadBeforeWriteMsg=warning  WriteAfterWriteMsg=warning  WriteAfterReadMsg=warning  ShowAdditionalParam=off  OutDataTypeStr=single
  Data Store Memory38 : DataStoreMemory  DataStoreName=AI06  ReadBeforeWriteMsg=warning  WriteAfterWriteMsg=warning  WriteAfterReadMsg=warning  ShowAdditionalParam=off  OutDataTypeStr=single
  Data Store Memory39 : DataStoreMemory  DataStoreName=AI07  ReadBeforeWriteMsg=warning  WriteAfterWriteMsg=warning  WriteAfterReadMsg=warning  ShowAdditionalParam=off  OutDataTypeStr=single
  Data Store Memory4 : DataStoreMemory  DataStoreName=Init_flg  ReadBeforeWriteMsg=warning  WriteAfterWriteMsg=warning  WriteAfterReadMsg=warning  ShowAdditionalParam=off  OutDataTypeStr=uint8
  Data Store Memory40 : DataStoreMemory  DataStoreName=AI08  ReadBeforeWriteMsg=warning  WriteAfterWriteMsg=warning  WriteAfterReadMsg=warning  ShowAdditionalParam=off  OutDataTypeStr=single
  Data Store Memory41 : DataStoreMemory  DataStoreName=AI12  ReadBeforeWriteMsg=warning  WriteAfterWriteMsg=warning  WriteAfterReadMsg=warning  ShowAdditionalParam=off  OutDataTypeStr=single
  Data Store Memory42 : DataStoreMemory  DataStoreName=AI15  ReadBeforeWriteMsg=warning  WriteAfterWriteMsg=warning  WriteAfterReadMsg=warning  ShowAdditionalParam=off  OutDataTypeStr=single
  Data Store Memory43 : DataStoreMemory  DataStoreName=AI17  ReadBeforeWriteMsg=warning  WriteAfterWriteMsg=warning  WriteAfterReadMsg=warning  ShowAdditionalParam=off  OutDataTypeStr=single
  Data Store Memory44 : DataStoreMemory  DataStoreName=AI04  ReadBeforeWriteMsg=warning  WriteAfterWriteMsg=warning  WriteAfterReadMsg=warning  ShowAdditionalParam=off  OutDataTypeStr=single
  Data Store Memory45 : DataStoreMemory  DataStoreName=LS017  ReadBeforeWriteMsg=warning  WriteAfterWriteMsg=warning  WriteAfterReadMsg=warning  ShowAdditionalParam=off  OutDataTypeStr=boolean
      settings: RTWStateStorageClass=ExportedGlobal
  Data Store Memory46 : DataStoreMemory  DataStoreName=Cnt_TW1  ReadBeforeWriteMsg=warning  WriteAfterWriteMsg=warning  WriteAfterReadMsg=warning  ShowAdditionalParam=off  OutDataTypeStr=uint8
      settings: RTWStateStorageClass=ExportedGlobal
  Data Store Memory47 : DataStoreMemory  DataStoreName=Cnt_TW2  ReadBeforeWriteMsg=warning  WriteAfterWriteMsg=warning  WriteAfterReadMsg=warning  ShowAdditionalParam=off  OutDataTypeStr=uint8
      settings: RTWStateStorageClass=ExportedGlobal
  Data Store Memory48 : DataStoreMemory  DataStoreName=Cnt_TW3  ReadBeforeWriteMsg=warning  WriteAfterWriteMsg=warning  WriteAfterReadMsg=warning  ShowAdditionalParam=off  OutDataTypeStr=uint8
      settings: RTWStateStorageClass=ExportedGlobal
  Data Store Memory49 : DataStoreMemory  DataStoreName=Cnt_ISG1  ReadBeforeWriteMsg=warning  WriteAfterWriteMsg=warning  WriteAfterReadMsg=warning  ShowAdditionalParam=off  OutDataTypeStr=uint8
      settings: RTWStateStorageClass=ExportedGlobal
  Data Store Memory5 : DataStoreMemory  DataStoreName=Cnt_BRS1  ReadBeforeWriteMsg=warning  WriteAfterWriteMsg=warning  WriteAfterReadMsg=warning  ShowAdditionalParam=off  OutDataTypeStr=uint8
      settings: RTWStateStorageClass=ExportedGlobal
  Data Store Memory50 : DataStoreMemory  DataStoreName=Cnt_ISG2  ReadBeforeWriteMsg=warning  WriteAfterWriteMsg=warning  WriteAfterReadMsg=warning  ShowAdditionalParam=off  OutDataTypeStr=uint8
      settings: RTWStateStorageClass=ExportedGlobal
  Data Store Memory51 : DataStoreMemory  DataStoreName=AI05  ReadBeforeWriteMsg=warning  WriteAfterWriteMsg=warning  WriteAfterReadMsg=warning  ShowAdditionalParam=off  OutDataTypeStr=single
  Data Store Memory52 : DataStoreMemory  DataStoreName=AI09  ReadBeforeWriteMsg=warning  WriteAfterWriteMsg=warning  WriteAfterReadMsg=warning  ShowAdditionalParam=off  OutDataTypeStr=single
  Data Store Memory53 : DataStoreMemory  DataStoreName=AI20  ReadBeforeWriteMsg=warning  WriteAfterWriteMsg=warning  WriteAfterReadMsg=warning  ShowAdditionalParam=off  OutDataTypeStr=single
  Data Store Memory54 : DataStoreMemory  DataStoreName=DI31  ReadBeforeWriteMsg=warning  WriteAfterWriteMsg=warning  WriteAfterReadMsg=warning  ShowAdditionalParam=off  OutDataTypeStr=boolean
  Data Store Memory55 : DataStoreMemory  DataStoreName=DI32  ReadBeforeWriteMsg=warning  WriteAfterWriteMsg=warning  WriteAfterReadMsg=warning  ShowAdditionalParam=off  OutDataTypeStr=boolean
  Data Store Memory56 : DataStoreMemory  DataStoreName=Cnt_ISG3  ReadBeforeWriteMsg=warning  WriteAfterWriteMsg=warning  WriteAfterReadMsg=warning  ShowAdditionalParam=off  OutDataTypeStr=uint8
      settings: RTWStateStorageClass=ExportedGlobal
  Data Store Memory57 : DataStoreMemory  DataStoreName=Cnt_BMS_OUT  ReadBeforeWriteMsg=warning  WriteAfterWriteMsg=warning  WriteAfterReadMsg=warning  ShowAdditionalParam=off  OutDataTypeStr=uint8
      settings: RTWStateStorageClass=ExportedGlobal
  Data Store Memory58 : DataStoreMemory  DataStoreName=Cnt_TMS_OUT  ReadBeforeWriteMsg=warning  WriteAfterWriteMsg=warning  WriteAfterReadMsg=warning  ShowAdditionalParam=off  OutDataTypeStr=uint8
      settings: RTWStateStorageClass=ExportedGlobal
  Data Store Memory59 : DataStoreMemory  DataStoreName=Cnt_ICU_OUT1  ReadBeforeWriteMsg=warning  WriteAfterWriteMsg=warning  WriteAfterReadMsg=warning  ShowAdditionalParam=off  OutDataTypeStr=uint8
      settings: RTWStateStorageClass=ExportedGlobal
  Data Store Memory6 : DataStoreMemory  DataStoreName=Cnt_BRS2  ReadBeforeWriteMsg=warning  WriteAfterWriteMsg=warning  WriteAfterReadMsg=warning  ShowAdditionalParam=off  OutDataTypeStr=uint8
      settings: RTWStateStorageClass=ExportedGlobal
  Data Store Memory60 : DataStoreMemory  DataStoreName=Cnt_ICU_OUT2  ReadBeforeWriteMsg=warning  WriteAfterWriteMsg=warning  WriteAfterReadMsg=warning  ShowAdditionalParam=off  OutDataTypeStr=uint8
      settings: RTWStateStorageClass=ExportedGlobal
  Data Store Memory61 : DataStoreMemory  DataStoreName=Cnt_BRS_OUT  ReadBeforeWriteMsg=warning  WriteAfterWriteMsg=warning  WriteAfterReadMsg=warning  ShowAdditionalParam=off  OutDataTypeStr=uint8
      settings: RTWStateStorageClass=ExportedGlobal
  Data Store Memory62 : DataStoreMemory  DataStoreName=Cnt_DCDC_OUT  ReadBeforeWriteMsg=warning  WriteAfterWriteMsg=warning  WriteAfterReadMsg=warning  ShowAdditionalParam=off  OutDataTypeStr=uint8
      settings: RTWStateStorageClass=ExportedGlobal
  Data Store Memory63 : DataStoreMemory  DataStoreName=Cnt_HVC_OUT  ReadBeforeWriteMsg=warning  WriteAfterWriteMsg=warning  WriteAfterReadMsg=warning  ShowAdditionalParam=off  OutDataTypeStr=uint8
      settings: RTWStateStorageClass=ExportedGlobal
  Data Store Memory64 : DataStoreMemory  DataStoreName=Cnt_MCU1_OUT  ReadBeforeWriteMsg=warning  WriteAfterWriteMsg=warning  WriteAfterReadMsg=warning  ShowAdditionalParam=off  OutDataTypeStr=uint8
      settings: RTWStateStorageClass=ExportedGlobal
  Data Store Memory65 : DataStoreMemory  DataStoreName=Cnt_ACU_OUT  ReadBeforeWriteMsg=warning  WriteAfterWriteMsg=warning  WriteAfterReadMsg=warning  ShowAdditionalParam=off  OutDataTypeStr=uint8
      settings: RTWStateStorageClass=ExportedGlobal
  Data Store Memory66 : DataStoreMemory  DataStoreName=Cnt_PDU_OUT  ReadBeforeWriteMsg=warning  WriteAfterWriteMsg=warning  WriteAfterReadMsg=warning  ShowAdditionalParam=off  OutDataTypeStr=uint8
      settings: RTWStateStorageClass=ExportedGlobal
  Data Store Memory67 : DataStoreMemory  DataStoreName=DI33  ReadBeforeWriteMsg=warning  WriteAfterWriteMsg=warning  WriteAfterReadMsg=warning  ShowAdditionalParam=off  OutDataTypeStr=boolean
  Data Store Memory68 : DataStoreMemory  DataStoreName=DI07  ReadBeforeWriteMsg=warning  WriteAfterWriteMsg=warning  WriteAfterReadMsg=warning  ShowAdditionalParam=off  OutDataTypeStr=boolean
  Data Store Memory69 : DataStoreMemory  DataStoreName=DI01  ReadBeforeWriteMsg=warning  WriteAfterWriteMsg=warning  WriteAfterReadMsg=warning  ShowAdditionalParam=off  OutDataTypeStr=boolean
  Data Store Memory7 : DataStoreMemory  DataStoreName=Cnt_BRS3  ReadBeforeWriteMsg=warning  WriteAfterWriteMsg=warning  WriteAfterReadMsg=warning  ShowAdditionalParam=off  OutDataTypeStr=uint8
      settings: RTWStateStorageClass=ExportedGlobal
  Data Store Memory70 : DataStoreMemory  DataStoreName=DI10  ReadBeforeWriteMsg=warning  WriteAfterWriteMsg=warning  WriteAfterReadMsg=warning  ShowAdditionalParam=off  OutDataTypeStr=boolean
  Data Store Memory71 : DataStoreMemory  DataStoreName=DI13  ReadBeforeWriteMsg=warning  WriteAfterWriteMsg=warning  WriteAfterReadMsg=warning  ShowAdditionalParam=off  OutDataTypeStr=boolean
  Data Store Memory72 : DataStoreMemory  DataStoreName=ResetFlg  ReadBeforeWriteMsg=warning  WriteAfterWriteMsg=warning  WriteAfterReadMsg=warning  ShowAdditionalParam=off  OutDataTypeStr=uint8
      settings: RTWStateStorageClass=ExportedGlobal
  Data Store Memory73 : DataStoreMemory  DataStoreName=DI15  ReadBeforeWriteMsg=warning  WriteAfterWriteMsg=warning  WriteAfterReadMsg=warning  ShowAdditionalParam=off  OutDataTypeStr=boolean
  Data Store Memory74 : DataStoreMemory  DataStoreName=DI16  ReadBeforeWriteMsg=warning  WriteAfterWriteMsg=warning  WriteAfterReadMsg=warning  ShowAdditionalParam=off  OutDataTypeStr=boolean
  Data Store Memory75 : DataStoreMemory  DataStoreName=DI17  ReadBeforeWriteMsg=warning  WriteAfterWriteMsg=warning  WriteAfterReadMsg=warning  ShowAdditionalParam=off  OutDataTypeStr=boolean
  Data Store Memory76 : DataStoreMemory  DataStoreName=DI18  ReadBeforeWriteMsg=warning  WriteAfterWriteMsg=warning  WriteAfterReadMsg=warning  ShowAdditionalParam=off  OutDataTypeStr=boolean
  Data Store Memory77 : DataStoreMemory  DataStoreName=DI02  ReadBeforeWriteMsg=warning  WriteAfterWriteMsg=warning  WriteAfterReadMsg=warning  ShowAdditionalParam=off  OutDataTypeStr=boolean
  Data Store Memory78 : DataStoreMemory  DataStoreName=DI03  ReadBeforeWriteMsg=warning  WriteAfterWriteMsg=warning  WriteAfterReadMsg=warning  ShowAdditionalParam=off  OutDataTypeStr=boolean
  Data Store Memory79 : DataStoreMemory  DataStoreName=DI34  ReadBeforeWriteMsg=warning  WriteAfterWriteMsg=warning  WriteAfterReadMsg=warning  ShowAdditionalParam=off  OutDataTypeStr=boolean
  Data Store Memory8 : DataStoreMemory  DataStoreName=Cnt_HVC1  ReadBeforeWriteMsg=warning  WriteAfterWriteMsg=warning  WriteAfterReadMsg=warning  ShowAdditionalParam=off  OutDataTypeStr=uint8
      settings: RTWStateStorageClass=ExportedGlobal
  Data Store Memory80 : DataStoreMemory  DataStoreName=DI04  ReadBeforeWriteMsg=warning  WriteAfterWriteMsg=warning  WriteAfterReadMsg=warning  ShowAdditionalParam=off  OutDataTypeStr=boolean
  Data Store Memory81 : DataStoreMemory  DataStoreName=DI12  ReadBeforeWriteMsg=warning  WriteAfterWriteMsg=warning  WriteAfterReadMsg=warning  ShowAdditionalParam=off  OutDataTypeStr=boolean
  Data Store Memory82 : DataStoreMemory  DataStoreName=DI08  ReadBeforeWriteMsg=warning  WriteAfterWriteMsg=warning  WriteAfterReadMsg=warning  ShowAdditionalParam=off  OutDataTypeStr=boolean
  Data Store Memory83 : DataStoreMemory  DataStoreName=LSO17_ETC_DC  ReadBeforeWriteMsg=warning  WriteAfterWriteMsg=warning  WriteAfterReadMsg=warning  ShowAdditionalParam=off  OutMin=0  OutMax=1  OutDataTypeStr=single
  Data Store Memory84 : DataStoreMemory  DataStoreName=DI09  ReadBeforeWriteMsg=warning  WriteAfterWriteMsg=warning  WriteAfterReadMsg=warning  ShowAdditionalParam=off  OutDataTypeStr=boolean
  Data Store Memory85 : DataStoreMemory  DataStoreName=HS014_ETC_DC  ReadBeforeWriteMsg=warning  WriteAfterWriteMsg=warning  WriteAfterReadMsg=warning  ShowAdditionalParam=off  OutMin=0  OutMax=1  OutDataTypeStr=single
  Data Store Memory86 : DataStoreMemory  DataStoreName=LS014  ReadBeforeWriteMsg=warning  WriteAfterWriteMsg=warning  WriteAfterReadMsg=warning  ShowAdditionalParam=off  OutDataTypeStr=boolean
      settings: RTWStateStorageClass=ExportedGlobal
  Data Store Memory87 : DataStoreMemory  DataStoreName=LS015  ReadBeforeWriteMsg=warning  WriteAfterWriteMsg=warning  WriteAfterReadMsg=warning  ShowAdditionalParam=off  OutDataTypeStr=boolean
      settings: RTWStateStorageClass=ExportedGlobal
  Data Store Memory88 : DataStoreMemory  DataStoreName=LS009  ReadBeforeWriteMsg=warning  WriteAfterWriteMsg=warning  WriteAfterReadMsg=warning  ShowAdditionalParam=off  OutDataTypeStr=boolean
      settings: RTWStateStorageClass=ExportedGlobal
  Data Store Memory89 : DataStoreMemory  DataStoreName=LS016  ReadBeforeWriteMsg=warning  WriteAfterWriteMsg=warning  WriteAfterReadMsg=warning  ShowAdditionalParam=off  OutDataTypeStr=boolean
      settings: RTWStateStorageClass=ExportedGlobal
  Data Store Memory9 : DataStoreMemory  DataStoreName=Cnt_HVC3  ReadBeforeWriteMsg=warning  WriteAfterWriteMsg=warning  WriteAfterReadMsg=warning  ShowAdditionalParam=off  OutDataTypeStr=uint8
      settings: RTWStateStorageClass=ExportedGlobal
  Data Store Memory90 : DataStoreMemory  DataStoreName=HS008_ETC_DC  ReadBeforeWriteMsg=warning  WriteAfterWriteMsg=warning  WriteAfterReadMsg=warning  ShowAdditionalParam=off  OutMin=0  OutMax=1  OutDataTypeStr=single
  Data Store Memory91 : DataStoreMemory  DataStoreName=LS004  ReadBeforeWriteMsg=warning  WriteAfterWriteMsg=warning  WriteAfterReadMsg=warning  ShowAdditionalParam=off  OutDataTypeStr=boolean
      settings: RTWStateStorageClass=ExportedGlobal
  Data Store Memory92 : DataStoreMemory  DataStoreName=LS011  ReadBeforeWriteMsg=warning  WriteAfterWriteMsg=warning  WriteAfterReadMsg=warning  ShowAdditionalParam=off  OutDataTypeStr=boolean
      settings: RTWStateStorageClass=ExportedGlobal
  Data Store Memory93 : DataStoreMemory  DataStoreName=LS001  ReadBeforeWriteMsg=warning  WriteAfterWriteMsg=warning  WriteAfterReadMsg=warning  ShowAdditionalParam=off  OutDataTypeStr=boolean
      settings: RTWStateStorageClass=ExportedGlobal
  Data Store Memory94 : DataStoreMemory  DataStoreName=HS006  ReadBeforeWriteMsg=warning  WriteAfterWriteMsg=warning  WriteAfterReadMsg=warning  ShowAdditionalParam=off  OutDataTypeStr=boolean
  Data Store Memory95 : DataStoreMemory  DataStoreName=LS002  ReadBeforeWriteMsg=warning  WriteAfterWriteMsg=warning  WriteAfterReadMsg=warning  ShowAdditionalParam=off  OutDataTypeStr=boolean
      settings: RTWStateStorageClass=ExportedGlobal
  Data Store Memory96 : DataStoreMemory  DataStoreName=LS010  ReadBeforeWriteMsg=warning  WriteAfterWriteMsg=warning  WriteAfterReadMsg=warning  ShowAdditionalParam=off  OutDataTypeStr=boolean
      settings: RTWStateStorageClass=ExportedGlobal
  Data Store Memory97 : DataStoreMemory  DataStoreName=LS008  ReadBeforeWriteMsg=warning  WriteAfterWriteMsg=warning  WriteAfterReadMsg=warning  ShowAdditionalParam=off  OutDataTypeStr=boolean
      settings: RTWStateStorageClass=ExportedGlobal
  Data Store Memory98 : DataStoreMemory  DataStoreName=Init_flg_SPI  ReadBeforeWriteMsg=warning  WriteAfterWriteMsg=warning  WriteAfterReadMsg=warning  ShowAdditionalParam=off  OutDataTypeStr=uint8
      settings: RTWStateStorageClass=ExportedGlobal
  Data Store Memory99 : DataStoreMemory  DataStoreName=LS006  ReadBeforeWriteMsg=warning  WriteAfterWriteMsg=warning  WriteAfterReadMsg=warning  ShowAdditionalParam=off  OutDataTypeStr=boolean
      settings: RTWStateStorageClass=ExportedGlobal
  Data Store Read : DataStoreRead  Commented=on  DataStoreName=HS004
  Data Store Read1 : DataStoreRead  DataStoreName=AI09
  Data Store Write1 : DataStoreWrite  Commented=on  DataStoreName=LS006
  Data Store Write10 : DataStoreWrite  Commented=on  DataStoreName=LS013
  Data Store Write11 : DataStoreWrite  Commented=on  DataStoreName=LS002
  Data Store Write12 : DataStoreWrite  Commented=on  DataStoreName=LS004
  Data Store Write2 : DataStoreWrite  Commented=on  DataStoreName=LS007
  Data Store Write3 : DataStoreWrite  Commented=on  DataStoreName=LS008
  Data Store Write5 : DataStoreWrite  Commented=on  DataStoreName=HS007
  Data Store Write6 : DataStoreWrite  Commented=on  DataStoreName=HS010
  Data Store Write7 : DataStoreWrite  Commented=on  DataStoreName=HS006
  Data Store Write8 : DataStoreWrite  Commented=on  DataStoreName=LS010
  Data Store Write9 : DataStoreWrite  Commented=on  DataStoreName=LS012
  FCAN_Config4 : mbd_mpc574x_ec_toolbox/Communication Blocks/CAN Blocks/FCAN_Config  Priority=1  can_instance=0  can_mode=Normal mode  can_max_num_mb=63  can_rx=PTB1: [CAN0_RX | CAN 0 Receive Pin]  can_tx=PTB0: [CAN0_TX | CAN 0 Transmit Pin]  show_adv_opts=on  can_clk_src=Peripheral clock  bitrate_to_time_seg=on  bitrate=250  sample_point=87.5  can_presdiv=18  can_propseg=7  can_pseg1=2  can_pseg2=1  can_rjw=2  cbt_bitrate=1000  cbt_sample_point=87.5  can_cbt_presdiv=1  can_cbt_propseg=6  can_cbt_pseg1=7  can_cbt_pseg2=7  can_cbt_rjw=3  can_fd_enable=off  can_payload=8  can_rxfifo_enable=off  can_fifo_id_filter_extended=off  can_fifo_id_filter_remote=off  can_num_id_filters=8  can_fifo_id_format=A  can_fifo_id_filter={'0x0', '0x0', '0x0', '0x0', '0x0', '0x0', '0x0', '0x0'}  can_pn_enable=off  can_wakeup_match=off  can_wakeup_timeout=off  can_timeout_en=off  can_match_timeout=1  can_multiple_matches_en=off  can_num_matches=1  can_idfilter_extendedid=off  can_idfilter_remoteframe=off  can_idfilter_type=Match exact  can_idfilter_id1=0  can_idfilter_id2=0  can_payloadfilter_enable=off  can_payloadfilter_dlclow=0  can_payloadfilter_dlchigh=0  can_payloadfilter_type=Match exact  can_payloadfilter_payload1_b0=0  can_payloadfilter_payload1_b1=0  can_payloadfilter_payload1_b2=0  can_payloadfilter_payload1_b3=0  can_payloadfilter_payload1_b4=0  can_payloadfilter_payload1_b5=0  can_payloadfilter_payload1_b6=0  can_payloadfilter_payload1_b7=0  can_payloadfilter_payload2_b0=0  can_payloadfilter_payload2_b1=0  can_payloadfilter_payload2_b2=0  can_payloadfilter_payload2_b3=0  can_payloadfilter_payload2_b4=0  can_payloadfilter_payload2_b5=0  can_payloadfilter_payload2_b6=0  can_payloadfilter_payload2_b7=0
  FCAN_Config5 : mbd_mpc574x_ec_toolbox/Communication Blocks/CAN Blocks/FCAN_Config  Priority=1  Commented=on  can_instance=2  can_mode=Normal mode  can_max_num_mb=63  can_rx=PTF15: [CAN2_RX | CAN2 RXD]  can_tx=PTF14: [CAN2_TX | CAN 2 Transmit Pin]  show_adv_opts=on  can_clk_src=Peripheral clock  bitrate_to_time_seg=on  bitrate=500  sample_point=87.5  can_presdiv=6  can_propseg=7  can_pseg1=6  can_pseg2=2  can_rjw=3  cbt_bitrate=1000  cbt_sample_point=87.5  can_cbt_presdiv=1  can_cbt_propseg=6  can_cbt_pseg1=7  can_cbt_pseg2=7  can_cbt_rjw=3  can_fd_enable=off  can_payload=8  can_rxfifo_enable=off  can_fifo_id_filter_extended=off  can_fifo_id_filter_remote=off  can_num_id_filters=8  can_fifo_id_format=A  can_fifo_id_filter={'0x0', '0x0', '0x0', '0x0', '0x0', '0x0', '0x0', '0x0'}  can_pn_enable=off  can_wakeup_match=off  can_wakeup_timeout=off  can_timeout_en=off  can_match_timeout=1  can_multiple_matches_en=off  can_num_matches=1  can_idfilter_extendedid=off  can_idfilter_remoteframe=off  can_idfilter_type=Match exact  can_idfilter_id1=0  can_idfilter_id2=0  can_payloadfilter_enable=off  can_payloadfilter_dlclow=0  can_payloadfilter_dlchigh=0  can_payloadfilter_type=Match exact  can_payloadfilter_payload1_b0=0  can_payloadfilter_payload1_b1=0  can_payloadfilter_payload1_b2=0  can_payloadfilter_payload1_b3=0  can_payloadfilter_payload1_b4=0  can_payloadfilter_payload1_b5=0  can_payloadfilter_payload1_b6=0  can_payloadfilter_payload1_b7=0  can_payloadfilter_payload2_b0=0  can_payloadfilter_payload2_b1=0  can_payloadfilter_payload2_b2=0  can_payloadfilter_payload2_b3=0  can_payloadfilter_payload2_b4=0  can_payloadfilter_payload2_b5=0  can_payloadfilter_payload2_b6=0  can_payloadfilter_payload2_b7=0
  FCAN_Config6 : mbd_mpc574x_ec_toolbox/Communication Blocks/CAN Blocks/FCAN_Config  Priority=1  can_instance=1  can_mode=Normal mode  can_max_num_mb=63  can_rx=PTA15: [CAN1_RX | CAN 1 Receive Pin]  can_tx=PTA14: [CAN1_TX | CAN 1 Transmit Pin]  show_adv_opts=on  can_clk_src=Peripheral clock  bitrate_to_time_seg=on  bitrate=250  sample_point=87.5  can_presdiv=18  can_propseg=7  can_pseg1=2  can_pseg2=1  can_rjw=2  cbt_bitrate=1000  cbt_sample_point=87.5  can_cbt_presdiv=1  can_cbt_propseg=6  can_cbt_pseg1=7  can_cbt_pseg2=7  can_cbt_rjw=3  can_fd_enable=off  can_payload=8  can_rxfifo_enable=off  can_fifo_id_filter_extended=off  can_fifo_id_filter_remote=off  can_num_id_filters=8  can_fifo_id_format=A  can_fifo_id_filter={'0x0', '0x0', '0x0', '0x0', '0x0', '0x0', '0x0', '0x0'}  can_pn_enable=off  can_wakeup_match=off  can_wakeup_timeout=off  can_timeout_en=off  can_match_timeout=1  can_multiple_matches_en=off  can_num_matches=1  can_idfilter_extendedid=off  can_idfilter_remoteframe=off  can_idfilter_type=Match exact  can_idfilter_id1=0  can_idfilter_id2=0  can_payloadfilter_enable=off  can_payloadfilter_dlclow=0  can_payloadfilter_dlchigh=0  can_payloadfilter_type=Match exact  can_payloadfilter_payload1_b0=0  can_payloadfilter_payload1_b1=0  can_payloadfilter_payload1_b2=0  can_payloadfilter_payload1_b3=0  can_payloadfilter_payload1_b4=0  can_payloadfilter_payload1_b5=0  can_payloadfilter_payload1_b6=0  can_payloadfilter_payload1_b7=0  can_payloadfilter_payload2_b0=0  can_payloadfilter_payload2_b1=0  can_payloadfilter_payload2_b2=0  can_payloadfilter_payload2_b3=0  can_payloadfilter_payload2_b4=0  can_payloadfilter_payload2_b5=0  can_payloadfilter_payload2_b6=0  can_payloadfilter_payload2_b7=0
  FreeMaster_Config : mbd_mpc574x_ec_toolbox/Utility Blocks/FreeMaster_Config  interface=CAN2  baudrate=500K  rxd=PTF15: [CAN2_RX | CAN2 RXD]  txd=PTF14: [CAN2_TX | CAN 2 Transmit Pin]  mode=Poll-driven  isr_prio=15  show_adv_opts=on  use_scope=on  max_scope_vars=8  use_recorder=on  max_rec_vars=8  rec_buff_size=1024  rec_timebase=0 seconds  comm_buffer_size_auto=on  comm_buffer_size=255  comm_rqueue_size_default=on  comm_rqueue_size=32
  Init : Subsystem  TreatAsAtomicUnit=on
  Initialization & SPI timer1 : Subsystem
  MBD_MPC574x_Config_Information1 : mbd_mpc574x_ec_toolbox/MBD_MPC574x_Config_Information  Priority=0  disp_str=|  config_params=[]  mcu_target_name=MPC5744P  mcu_target_package=144-LQFP  mcu_target_sram_size=384KB  mcu_system_clock_freq=200  mcu_xtal_freq=40  mcu_step_timer=PIT Channel 0  mcu_step_priority=1  ds_import_enable=on  target_compiler=S32 Design Studio  target_memory=FLASH  s32ds_target_compile_opts=-g3 -mbig -mvle -O1 -mregnames -mlsp -specs=ewl_c9x.specs -mhard-float -Wall -c -std=c99 -fdata-sections -ffunction-sections -funsigned-char -fmessage-length=0 -nostdinc -fno-jump-tables  s32ds_target_assemble_opts=-g3 -mbig -mvle -mregnames  s32ds_target_link_opts=-Xlinker --gc-sections -mhard-float  s32ds_target_default_lcf=on  s32ds_target_user_lcf=MPC5744P_flash.ld  ghs_target_compile_opts=-preprocess_assembly_files -g -dwarf2 -noSPE -filetype.c  ghs_target_assemble_opts=-preprocess_assembly_files -g -dwarf2 -e _start_core -srec -filetype.assembly  ghs_target_default_lcf=on  ghs_target_user_lcf=MPC5744P_flash.ld  diab_target_compile_opts=-@E+err.log -c -g -Xenum-is-best -Xlint -Xnested-interrupts -Xdebug-local-cie -Xclib-optim-off -Xc-new  diab_target_assemble_opts=-@E+err.log -l -g  diab_target_link_opts=-@E+err.log -Ws -m6 -lc -lm  diab_target_default_lcf=on  diab_target_user_lcf=MPC5744P_flash.dld  pil_download_enable=off  rbl_download_enable=on  rbl_start_delay=5000  rbl_restart_request=on  rbl_com_port=Custom  rbl_com_port_custom=COM1  pil_download_rate=115200  pil_interface=Serial 0  pil_rx=PTB3: [LIN0_RX | LIN 0 Receive Pin]  pil_tx=PTB2: [LIN0_TX | LINFlexD 0 Transmit Pin]  rbl_def_password=on  rbl_password=0xFEEDFACECAFEBEEF  rbl_manual_len_size=off  rbl_start_address=0  rbl_code_size=0  ADC_PcrCheckEnDis=on  FlexPWM_PcrCheckEnDis=off  CTU_PcrCheckEnDis=on  SWG_PcrCheckEnDis=on  eTimer_PcrCheckEnDis=off  EQADC_PcrCheckEnDis=on  eMIOS_PcrCheckEnDis=on  FlexCAN_PcrCheckEnDis=on  I2C_PcrCheckEnDis=on  MCAN_PcrCheckEnDis=on  SPI_PcrCheckEnDis=on  UART_PcrCheckEnDis=on  GPIO_OutputPcrCheckEnDis=on  GPIO_InputPcrCheckEnDis=on  eDMA_PcrCheckEnDis=on  PIT_PcrCheckEnDis=on  AMMCLIB_PcrCheckEnDis=on  FM_PcrCheckEnDis=on  Profiler_PcrCheckEnDis=on  ModelRef_PcrCheckEnDis=on  ModelPinCheck_PcrCheckEnDis=on
      | System Clock : 200 MHz
      | Target : MPC5744P
      | Package : 144LQFP
      | XTAL Freq : 40 MHz
      | Compiler : S32 Design Studio
      | Target Type : FLASH
      | Global Interrupt Priority : 8
      | System Tick Interrupt Priority : 12
      | Freemaster : None;
      | Download Code after build : off
  Power Managment : Subsystem
  SPI_Config_CANB&LS : mbd_mpc574x_ec_toolbox/Communication Blocks/SPI Blocks/SPI_Config  InstanceNumber=3  Role=Master  BaudRate=500000  ShowAdvanced=on  sin=PTE15: [DSPI3_SIN | DSPI 3 Serial Data Input]  sout=PTE14: [DSPI3_SOUT | DSPI 3 Serial Data Out]  sck=PTE13: [DSPI3_SCK | DSPI 3 Input/Output Serial Clock]  pcs0=None  pcs1=None  pcs2=PTD12: [DSPI3_CS2 | DSPI 3 Peripheral Chip Select 2]  pcs3=PTD14: [DSPI3_CS3 | DSPI 3 Peripheral Chip Select 3]  pcs4=None  pcs5=None  pcs6=None  pcs7=None  CPHA=DSPI_CLOCK_PHASE_2ND_EDGE  CPOL=DSPI_ACTIVE_HIGH  BitOrder=MSB first  TransferSize=16  WhichPCS=0  PCSPol=DSPI_ACTIVE_LOW  ContinuousTransfer=on
  SPI_Config_EEPROM&LS : mbd_mpc574x_ec_toolbox/Communication Blocks/SPI Blocks/SPI_Config  InstanceNumber=0  Role=Master  BaudRate=500000  ShowAdvanced=on  sin=PTC7: [DSPI0_SIN | DSPI 0 Serial Data Input]  sout=PTC6: [DSPI0_SOUT | DSPI 0 Serial Data Out]  sck=PTC5: [DSPI0_SCK | DSPI 0 Input/Output Serial Clock]  pcs0=PTC4: [DSPI0_CS0 | DSPI 0 Peripheral Chip Select 0]  pcs1=PTG8: [DSPI0_CS1 | DSPI 0 Peripheral Chip Select 1]  pcs2=None  pcs3=None  pcs4=None  pcs5=PTD8: [DSPI0_CS5 | DSPI 0 Peripheral Chip Select 5]  pcs6=None  pcs7=None  CPHA=DSPI_CLOCK_PHASE_2ND_EDGE  CPOL=DSPI_ACTIVE_HIGH  BitOrder=MSB first  TransferSize=16  WhichPCS=0  PCSPol=DSPI_ACTIVE_LOW  ContinuousTransfer=on
  SPI_EEPROM : Subsystem  Commented=on
  SigIn : Subsystem
  SigOut : Subsystem
  VehCtrl : Subsystem  Commented=on
  eTimer_Config : mbd_mpc574x_ec_toolbox/Motor Control Blocks/eTIMER Blocks/eTimer_Config  etimerModule=0  etimerChannel=2  etimerMode=COUNT Mode  etimerCountOnce=Count repeatedly  etimerCountLength=Continue counting to roll over  etimerCountDirection=Count up  etimerCountStart=on  etimerCaptureArm=on  etimerShowAdv=on  etimerPrimarySource=IP Bus clock divide by 32 prescaler  etimerPrimaryPolarity=True polarity  etimerSecondarySource=Counter 0 input pin  etimerSecondaryPolarity=True polarity  etimerSampleCount=Require 3 consecutive samples to be of equal value  etimerSamplePeriod=0  etimerOutEnable=The external pin is configured as an input  etimerOutPolarity=True polarity  etimerOutMode=Toggle OFLAG output using alternating compare registers  etimerCompMode="COMP1 and COMP2  are used when the counter is counting up"  etimerCompLoad1=COMP1 is never preload  etimerCompLoad2=COMP2 is never preload  etimerCapt1=Capture rising edges  etimerCapt2=Capture falling edges  etimerOneShot=Free running mode is selected  etimerMasterMode=Disable broadcast of this channel output  etimerCoForce=Other channels cannot force this channel output  etimerCoChanInit=Other channels cannot force re-initialization of this channel  etimerRedundant=off  etimerCOMP1init=0  etimerCOMP2init=0  etimerCNTRinit=0  etimerCh0=None  etimerCh1=None  etimerCh2=PTF0: [eTimer0_ETC2 | eTimer_0 Input Data Channel 2]  etimerCh3=None  etimerCh4=None  etimerCh5=None  etimerIsrTCFIE=off  etimerIsrTCF1IE=off  etimerIsrTCF2IE=off  etimerIsrTOFIE=off  etimerIsrIELFIE=off  etimerIsrIEHFIE=off  etimerIsrICF1IE=off  etimerIsrICF2IE=on  etimerIsrRCF=off  etimerIsrWDF=off
  eTimer_Config1 : mbd_mpc574x_ec_toolbox/Motor Control Blocks/eTIMER Blocks/eTimer_Config  etimerModule=1  etimerChannel=2  etimerMode=COUNT Mode  etimerCountOnce=Count repeatedly  etimerCountLength=Continue counting to roll over  etimerCountDirection=Count up  etimerCountStart=on  etimerCaptureArm=on  etimerShowAdv=on  etimerPrimarySource=IP Bus clock divide by 32 prescaler  etimerPrimaryPolarity=True polarity  etimerSecondarySource=Counter 0 input pin  etimerSecondaryPolarity=True polarity  etimerSampleCount=Require 3 consecutive samples to be of equal value  etimerSamplePeriod=0  etimerOutEnable=The external pin is configured as an input  etimerOutPolarity=True polarity  etimerOutMode=Toggle OFLAG output using alternating compare registers  etimerCompMode="COMP1 and COMP2  are used when the counter is counting up"  etimerCompLoad1=COMP1 is never preload  etimerCompLoad2=COMP2 is never preload  etimerCapt1=Capture rising edges  etimerCapt2=Capture falling edges  etimerOneShot=Free running mode is selected  etimerMasterMode=Disable broadcast of this channel output  etimerCoForce=Other channels cannot force this channel output  etimerCoChanInit=Other channels cannot force re-initialization of this channel  etimerRedundant=off  etimerCOMP1init=0  etimerCOMP2init=0  etimerCNTRinit=0  etimerCh0=None  etimerCh1=None  etimerCh2=PTD1: [eTimer1_ETC2 | eTimer_1 Input Data Channel 2]  etimerCh3=None  etimerCh4=None  etimerCh5=None  etimerIsrTCFIE=off  etimerIsrTCF1IE=off  etimerIsrTCF2IE=off  etimerIsrTOFIE=off  etimerIsrIELFIE=off  etimerIsrIEHFIE=off  etimerIsrICF1IE=off  etimerIsrICF2IE=on  etimerIsrRCF=off  etimerIsrWDF=off
  eTimer_Config10 : mbd_mpc574x_ec_toolbox/Motor Control Blocks/eTIMER Blocks/eTimer_Config  etimerModule=0  etimerChannel=3  etimerMode=COUNT Mode  etimerCountOnce=Count repeatedly  etimerCountLength=Count until compare and then reinitialize  etimerCountDirection=Count up  etimerCountStart=off  etimerCaptureArm=off  etimerShowAdv=on  etimerPrimarySource=IP Bus clock divide by 64 prescaler  etimerPrimaryPolarity=True polarity  etimerSecondarySource=Counter 0 input pin  etimerSecondaryPolarity=True polarity  etimerSampleCount=Require 3 consecutive samples to be of equal value  etimerSamplePeriod=0  etimerOutEnable=OFLAG output signal will be driven on the external pin  etimerOutPolarity=True polarity  etimerOutMode=Toggle OFLAG output using alternating compare registers  etimerCompMode="COMP1 and COMP2  are used when the counter is counting up"  etimerCompLoad1=Load COMP1 with CMPLD1 upon successful compare with the value in COMP2  etimerCompLoad2=Load COMP2 with CMPLD2 upon successful compare with the value in COMP2  etimerCapt1=Capture disabled  etimerCapt2=Capture disabled  etimerOneShot=Free running mode is selected  etimerMasterMode=Enable broadcast of this channel output  etimerCoForce=Other channels cannot force this channel output  etimerCoChanInit=Other channels cannot force re-initialization of this channel  etimerRedundant=off  etimerCOMP1init=3750  etimerCOMP2init=3750  etimerCNTRinit=1  etimerCh0=None  etimerCh1=None  etimerCh2=None  etimerCh3=PTA3: [eTimer0_ETC3 | eTimer_0 Input/Output Data Channel 3]  etimerCh4=None  etimerCh5=None  etimerIsrTCFIE=off  etimerIsrTCF1IE=off  etimerIsrTCF2IE=on  etimerIsrTOFIE=off  etimerIsrIELFIE=off  etimerIsrIEHFIE=off  etimerIsrICF1IE=off  etimerIsrICF2IE=off  etimerIsrRCF=off  etimerIsrWDF=off
  eTimer_Config11 : mbd_mpc574x_ec_toolbox/Motor Control Blocks/eTIMER Blocks/eTimer_Config  etimerModule=0  etimerChannel=5  etimerMode=COUNT Mode  etimerCountOnce=Count repeatedly  etimerCountLength=Count until compare and then reinitialize  etimerCountDirection=Count up  etimerCountStart=off  etimerCaptureArm=off  etimerShowAdv=on  etimerPrimarySource=IP Bus clock divide by 64 prescaler  etimerPrimaryPolarity=True polarity  etimerSecondarySource=Counter 0 input pin  etimerSecondaryPolarity=True polarity  etimerSampleCount=Require 3 consecutive samples to be of equal value  etimerSamplePeriod=0  etimerOutEnable=OFLAG output signal will be driven on the external pin  etimerOutPolarity=True polarity  etimerOutMode=Toggle OFLAG output using alternating compare registers  etimerCompMode="COMP1 and COMP2  are used when the counter is counting up"  etimerCompLoad1=Load COMP1 with CMPLD1 upon successful compare with the value in COMP2  etimerCompLoad2=Load COMP2 with CMPLD2 upon successful compare with the value in COMP2  etimerCapt1=Capture disabled  etimerCapt2=Capture disabled  etimerOneShot=Free running mode is selected  etimerMasterMode=Enable broadcast of this channel output  etimerCoForce=Other channels cannot force this channel output  etimerCoChanInit=Other channels cannot force re-initialization of this channel  etimerRedundant=off  etimerCOMP1init=3750  etimerCOMP2init=3750  etimerCNTRinit=1  etimerCh0=None  etimerCh1=None  etimerCh2=None  etimerCh3=None  etimerCh4=None  etimerCh5=PTC12: [eTimer0_ETC5 | eTimer_0 Input/Output Data Channel 5]  etimerIsrTCFIE=off  etimerIsrTCF1IE=off  etimerIsrTCF2IE=on  etimerIsrTOFIE=off  etimerIsrIELFIE=off  etimerIsrIEHFIE=off  etimerIsrICF1IE=off  etimerIsrICF2IE=off  etimerIsrRCF=off  etimerIsrWDF=off
  eTimer_Config12 : mbd_mpc574x_ec_toolbox/Motor Control Blocks/eTIMER Blocks/eTimer_Config  etimerModule=2  etimerChannel=2  etimerMode=COUNT Mode  etimerCountOnce=Count repeatedly  etimerCountLength=Count until compare and then reinitialize  etimerCountDirection=Count up  etimerCountStart=off  etimerCaptureArm=off  etimerShowAdv=on  etimerPrimarySource=IP Bus clock divide by 64 prescaler  etimerPrimaryPolarity=True polarity  etimerSecondarySource=Counter 0 input pin  etimerSecondaryPolarity=True polarity  etimerSampleCount=Require 3 consecutive samples to be of equal value  etimerSamplePeriod=0  etimerOutEnable=OFLAG output signal will be driven on the external pin  etimerOutPolarity=True polarity  etimerOutMode=Toggle OFLAG output using alternating compare registers  etimerCompMode="COMP1 and COMP2  are used when the counter is counting up"  etimerCompLoad1=Load COMP1 with CMPLD1 upon successful compare with the value in COMP2  etimerCompLoad2=Load COMP2 with CMPLD2 upon successful compare with the value in COMP2  etimerCapt1=Capture disabled  etimerCapt2=Capture disabled  etimerOneShot=Free running mode is selected  etimerMasterMode=Enable broadcast of this channel output  etimerCoForce=Other channels cannot force this channel output  etimerCoChanInit=Other channels cannot force re-initialization of this channel  etimerRedundant=off  etimerCOMP1init=3750  etimerCOMP2init=3750  etimerCNTRinit=1  etimerCh0=None  etimerCh1=None  etimerCh2=PTJ8: [eTimer2_ETC2 | eTimer_2 Input/Output Data Channel 2]  etimerCh3=None  etimerCh4=None  etimerCh5=None  etimerIsrTCFIE=off  etimerIsrTCF1IE=off  etimerIsrTCF2IE=on  etimerIsrTOFIE=off  etimerIsrIELFIE=off  etimerIsrIEHFIE=off  etimerIsrICF1IE=off  etimerIsrICF2IE=off  etimerIsrRCF=off  etimerIsrWDF=off
  eTimer_Config13 : mbd_mpc574x_ec_toolbox/Motor Control Blocks/eTIMER Blocks/eTimer_Config  Commented=on  etimerModule=1  etimerChannel=0  etimerMode=COUNT Mode  etimerCountOnce=Count repeatedly  etimerCountLength=Continue counting to roll over  etimerCountDirection=Count up  etimerCountStart=on  etimerCaptureArm=on  etimerShowAdv=on  etimerPrimarySource=IP Bus clock divide by 64 prescaler  etimerPrimaryPolarity=True polarity  etimerSecondarySource=Counter 0 input pin  etimerSecondaryPolarity=True polarity  etimerSampleCount=Require 3 consecutive samples to be of equal value  etimerSamplePeriod=0  etimerOutEnable=The external pin is configured as an input  etimerOutPolarity=True polarity  etimerOutMode=Toggle OFLAG output using alternating compare registers  etimerCompMode="COMP1 and COMP2  are used when the counter is counting up"  etimerCompLoad1=COMP1 is never preload  etimerCompLoad2=COMP2 is never preload  etimerCapt1=Capture rising edges  etimerCapt2=Capture falling edges  etimerOneShot=Free running mode is selected  etimerMasterMode=Disable broadcast of this channel output  etimerCoForce=Other channels cannot force this channel output  etimerCoChanInit=Other channels cannot force re-initialization of this channel  etimerRedundant=off  etimerCOMP1init=0  etimerCOMP2init=0  etimerCNTRinit=0  etimerCh0=PTC15: [eTimer1_ETC0 | eTimer_1 Input Data Channel 0]  etimerCh1=None  etimerCh2=None  etimerCh3=None  etimerCh4=None  etimerCh5=None  etimerIsrTCFIE=off  etimerIsrTCF1IE=off  etimerIsrTCF2IE=off  etimerIsrTOFIE=off  etimerIsrIELFIE=off  etimerIsrIEHFIE=off  etimerIsrICF1IE=off  etimerIsrICF2IE=on  etimerIsrRCF=off  etimerIsrWDF=off
  eTimer_Config2 : mbd_mpc574x_ec_toolbox/Motor Control Blocks/eTIMER Blocks/eTimer_Config  etimerModule=1  etimerChannel=3  etimerMode=COUNT Mode  etimerCountOnce=Count repeatedly  etimerCountLength=Continue counting to roll over  etimerCountDirection=Count up  etimerCountStart=on  etimerCaptureArm=on  etimerShowAdv=on  etimerPrimarySource=IP Bus clock divide by 32 prescaler  etimerPrimaryPolarity=True polarity  etimerSecondarySource=Counter 0 input pin  etimerSecondaryPolarity=True polarity  etimerSampleCount=Require 3 consecutive samples to be of equal value  etimerSamplePeriod=0  etimerOutEnable=The external pin is configured as an input  etimerOutPolarity=True polarity  etimerOutMode=Toggle OFLAG output using alternating compare registers  etimerCompMode="COMP1 and COMP2  are used when the counter is counting up"  etimerCompLoad1=COMP1 is never preload  etimerCompLoad2=COMP2 is never preload  etimerCapt1=Capture rising edges  etimerCapt2=Capture falling edges  etimerOneShot=Free running mode is selected  etimerMasterMode=Disable broadcast of this channel output  etimerCoForce=Other channels cannot force this channel output  etimerCoChanInit=Other channels cannot force re-initialization of this channel  etimerRedundant=off  etimerCOMP1init=0  etimerCOMP2init=0  etimerCNTRinit=0  etimerCh0=None  etimerCh1=None  etimerCh2=None  etimerCh3=PTD2: [eTimer1_ETC3 | eTimer_1 Input Data Channel 3]  etimerCh4=None  etimerCh5=None  etimerIsrTCFIE=off  etimerIsrTCF1IE=off  etimerIsrTCF2IE=off  etimerIsrTOFIE=off  etimerIsrIELFIE=off  etimerIsrIEHFIE=off  etimerIsrICF1IE=off  etimerIsrICF2IE=on  etimerIsrRCF=off  etimerIsrWDF=off
  eTimer_Config3 : mbd_mpc574x_ec_toolbox/Motor Control Blocks/eTIMER Blocks/eTimer_Config  etimerModule=1  etimerChannel=1  etimerMode=COUNT Mode  etimerCountOnce=Count repeatedly  etimerCountLength=Continue counting to roll over  etimerCountDirection=Count up  etimerCountStart=on  etimerCaptureArm=on  etimerShowAdv=on  etimerPrimarySource=IP Bus clock divide by 32 prescaler  etimerPrimaryPolarity=True polarity  etimerSecondarySource=Counter 0 input pin  etimerSecondaryPolarity=True polarity  etimerSampleCount=Require 3 consecutive samples to be of equal value  etimerSamplePeriod=0  etimerOutEnable=The external pin is configured as an input  etimerOutPolarity=True polarity  etimerOutMode=Toggle OFLAG output using alternating compare registers  etimerCompMode="COMP1 and COMP2  are used when the counter is counting up"  etimerCompLoad1=COMP1 is never preload  etimerCompLoad2=COMP2 is never preload  etimerCapt1=Capture rising edges  etimerCapt2=Capture falling edges  etimerOneShot=Free running mode is selected  etimerMasterMode=Disable broadcast of this channel output  etimerCoForce=Other channels cannot force this channel output  etimerCoChanInit=Other channels cannot force re-initialization of this channel  etimerRedundant=off  etimerCOMP1init=0  etimerCOMP2init=0  etimerCNTRinit=0  etimerCh0=None  etimerCh1=PTC13: [eTimer1_ETC1 | eTimer_1 Input Data Channel 1]  etimerCh2=None  etimerCh3=None  etimerCh4=None  etimerCh5=None  etimerIsrTCFIE=off  etimerIsrTCF1IE=off  etimerIsrTCF2IE=off  etimerIsrTOFIE=off  etimerIsrIELFIE=off  etimerIsrIEHFIE=off  etimerIsrICF1IE=off  etimerIsrICF2IE=on  etimerIsrRCF=off  etimerIsrWDF=off
  eTimer_Config8 : mbd_mpc574x_ec_toolbox/Motor Control Blocks/eTIMER Blocks/eTimer_Config  Commented=on  etimerModule=1  etimerChannel=4  etimerMode=COUNT Mode  etimerCountOnce=Count repeatedly  etimerCountLength=Count until compare and then reinitialize  etimerCountDirection=Count up  etimerCountStart=off  etimerCaptureArm=off  etimerShowAdv=on  etimerPrimarySource=IP Bus clock divide by 32 prescaler  etimerPrimaryPolarity=True polarity  etimerSecondarySource=Counter 0 input pin  etimerSecondaryPolarity=True polarity  etimerSampleCount=Require 3 consecutive samples to be of equal value  etimerSamplePeriod=0  etimerOutEnable=OFLAG output signal will be driven on the external pin  etimerOutPolarity=True polarity  etimerOutMode=Toggle OFLAG output using alternating compare registers  etimerCompMode="COMP1 and COMP2  are used when the counter is counting up"  etimerCompLoad1=Load COMP1 with CMPLD1 upon successful compare with the value in COMP2  etimerCompLoad2=Load COMP2 with CMPLD2 upon successful compare with the value in COMP2  etimerCapt1=Capture disabled  etimerCapt2=Capture disabled  etimerOneShot=Free running mode is selected  etimerMasterMode=Enable broadcast of this channel output  etimerCoForce=Other channels cannot force this channel output  etimerCoChanInit=Other channels cannot force re-initialization of this channel  etimerRedundant=off  etimerCOMP1init=3750  etimerCOMP2init=3750  etimerCNTRinit=1  etimerCh0=None  etimerCh1=None  etimerCh2=None  etimerCh3=None  etimerCh4=PTD3: [eTimer1_ETC4 | eTimer_1 Input/Output Data Channel 4]  etimerCh5=None  etimerIsrTCFIE=off  etimerIsrTCF1IE=off  etimerIsrTCF2IE=on  etimerIsrTOFIE=off  etimerIsrIELFIE=off  etimerIsrIEHFIE=off  etimerIsrICF1IE=off  etimerIsrICF2IE=off  etimerIsrRCF=off  etimerIsrWDF=off
  eTimer_Config9 : mbd_mpc574x_ec_toolbox/Motor Control Blocks/eTIMER Blocks/eTimer_Config  Commented=on  etimerModule=1  etimerChannel=5  etimerMode=COUNT Mode  etimerCountOnce=Count repeatedly  etimerCountLength=Count until compare and then reinitialize  etimerCountDirection=Count up  etimerCountStart=off  etimerCaptureArm=off  etimerShowAdv=on  etimerPrimarySource=IP Bus clock divide by 32 prescaler  etimerPrimaryPolarity=True polarity  etimerSecondarySource=Counter 0 input pin  etimerSecondaryPolarity=True polarity  etimerSampleCount=Require 3 consecutive samples to be of equal value  etimerSamplePeriod=0  etimerOutEnable=OFLAG output signal will be driven on the external pin  etimerOutPolarity=True polarity  etimerOutMode=Toggle OFLAG output using alternating compare registers  etimerCompMode="COMP1 and COMP2  are used when the counter is counting up"  etimerCompLoad1=Load COMP1 with CMPLD1 upon successful compare with the value in COMP2  etimerCompLoad2=Load COMP2 with CMPLD2 upon successful compare with the value in COMP2  etimerCapt1=Capture disabled  etimerCapt2=Capture disabled  etimerOneShot=Free running mode is selected  etimerMasterMode=Enable broadcast of this channel output  etimerCoForce=Other channels cannot force this channel output  etimerCoChanInit=Other channels cannot force re-initialization of this channel  etimerRedundant=off  etimerCOMP1init=3750  etimerCOMP2init=3750  etimerCNTRinit=1  etimerCh0=None  etimerCh1=None  etimerCh2=None  etimerCh3=None  etimerCh4=None  etimerCh5=PTD4: [eTimer1_ETC5 | eTimer_1 Input/Output Data Channel 5]  etimerIsrTCFIE=off  etimerIsrTCF1IE=off  etimerIsrTCF2IE=on  etimerIsrTOFIE=off  etimerIsrIELFIE=off  etimerIsrIEHFIE=off  etimerIsrICF1IE=off  etimerIsrICF2IE=off  etimerIsrRCF=off  etimerIsrWDF=off
  wires:
  Constant/1 -> Power Managment/1(PowerMode)
  SigIn/1(BMS) -> VehCtrl/1("BMS ")
  SigIn/2(OBC) -> VehCtrl/2("OBC ")
  SigIn/3(TMS) -> VehCtrl/3("TMS ")
  SigIn/5(MCU1) -> VehCtrl/5("MCU1 ")
  SigIn/6(MCU2) -> VehCtrl/6("MCU2 ")
  SigIn/7(HVC) -> VehCtrl/7("HVC ")
  SigIn/8(ACU) -> VehCtrl/8(ACU)
  SigIn/9(PDU) -> VehCtrl/9(PDU)
  SigIn/10(TWV) -> VehCtrl/10("TWV ")
  SigIn/11(TM) -> VehCtrl/11(TM)
  SigIn/12(ISG) -> VehCtrl/12("ISG ")
  SigIn/13(DCDC) -> VehCtrl/13("DCDC ")
  SigIn/14("DAQ ") -> VehCtrl/14("DAQ ")
  SigIn/4(BRS) -> VehCtrl/4(BRS)
  VehCtrl/1(BMS_OUT) -> SigOut/1(BMS_OUT)
  VehCtrl/2(DCDC_OUT) -> SigOut/2("DCDC_OUT ")
  VehCtrl/3(BRS_OUT) -> SigOut/3(BRS_OUT)
  VehCtrl/4(ICU) -> SigOut/4(ICU)
  VehCtrl/5(HVC_OUT) -> SigOut/5(HVC_OUT)
  VehCtrl/6(MCU1_OUT) -> SigOut/6(MCU_OUT1)
  VehCtrl/7(MCU2_OUT) -> SigOut/7(MCU_OUT2)
  VehCtrl/8(ACU_OUT) -> SigOut/8(ACU_OUT)
  VehCtrl/9(PDU_OUT) -> SigOut/9(PDU_OUT)
  VehCtrl/10(TM_OUT) -> SigOut/10(TM_OUT)
  VehCtrl/11(ISG_OUT) -> SigOut/11(ISG_OUT)
  VehCtrl/13(TWV_OUT) -> SigOut/13(TWV_OUT)
  VehCtrl/12("TMS_OUT ") -> SigOut/12(TMS_OUT)
